simulink model "PW_SMRv10"  (R2022b)
settings: Solver=VariableStepAuto  StartTime=0.0  StopTime=3600 * 5  RelTol=1e-3
libraries: nesl_utility x117, fl_lib x83, SimscapeFluids_lib x11, ee_lib x9, slpidlib x7, simulink x1
(part 1 of 2)
settings Model: Creator=cheap  LastModifiedBy=cheap

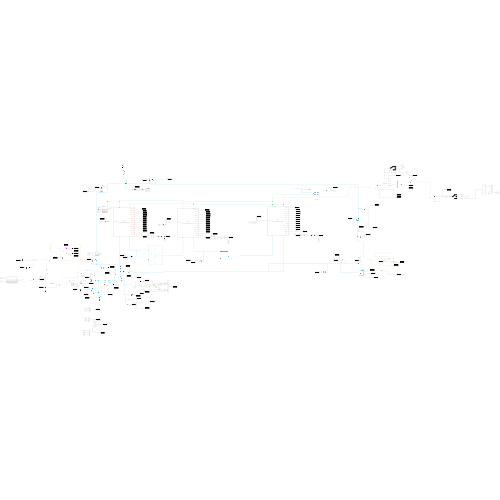
[thumbnail: Simulink's stored preview of the top-level diagram]
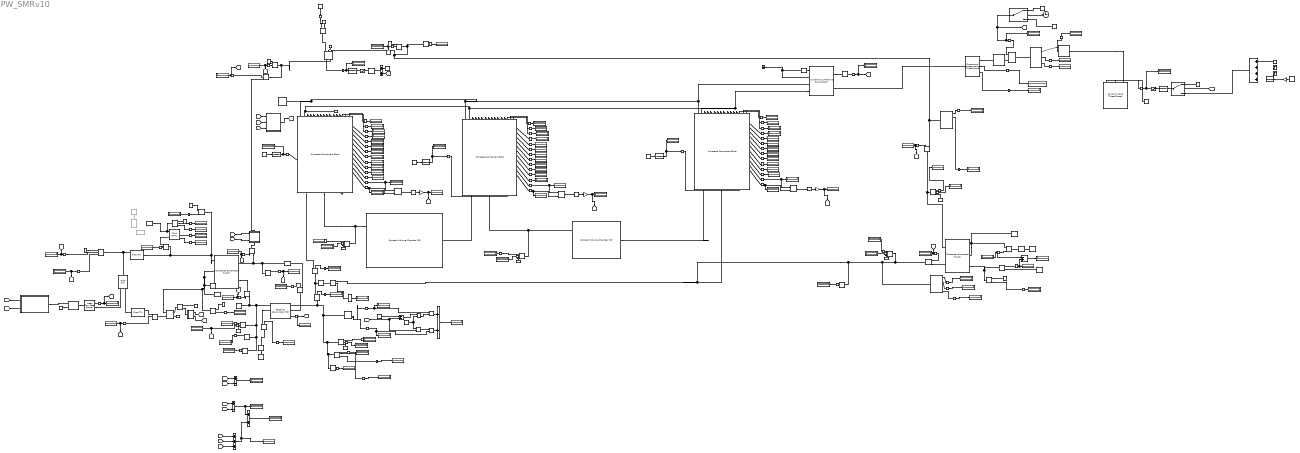
== system PW_SMRv10 ==
  Abs : Abs  SaturateOnIntegerOverflow=off
  Abs1 : Abs  SaturateOnIntegerOverflow=off
  Abs2 : Abs  SaturateOnIntegerOverflow=off
  Absolute Reference (2P){,1..7} (8 alike) : fl_lib/Two-Phase Fluid/Elements/Absolute Reference (2P)
  Absolute Reference (G) : fl_lib/Gas/Elements/Absolute Reference (G)
      settings: InternalSimscapePortConfiguration="{\"Bottom\":[],\"Left\":[{\"id\":\"A\",\"label\":\"\",\"type\":\"foundation.gas.gas\"}],\"Right\":[],\"Top\":[]}"
  Absolute Reference (TL){,1..3} (4 alike) : fl_lib/Thermal Liquid/Elements/Absolute Reference (TL)
  Add : Sum  Inputs=++++
  Add1 : Sum
  Add2 : Sum
  Add3 : Sum  Inputs=+++
  Band-Limited White Noise : simulink/Sources/Band-Limited White Noise  Cov=[0.01]  Ts=0.01  seed=[23341]
  Centrifugal Pump (TL) : SimscapeFluids_lib/Thermal Liquid/Pumps & Motors/Centrifugal Pump (TL)  pump_parameterization=fluids.thermal_liquid.pumps_motors.enum.CentrifugalPumpParameterization.Nominal  capacity_ref_nominal=1670 lpm  head_ref_nominal=40 m  power_ref_nominal=5.6 kW  head_ref_max=60 m  capacity_ref_max=2500 lpm  omega_ref_analytic=376.99 rad/s  flow_rate_1D_TLU=[16.67, 30, 40, 53.33, 66.67, 83.33] lpm  head_1D_TLU=[50, 47.5, 45, 40, 35, 25] m  power_1D_TLU=[.6, .75, .85, .93, .98, .99] kW  omega_ref_1D=3500 rpm  rho_ref_1D=998.21 kg/m^3  flow_rate_2D_TLU=[16.67, 23.33, 30, 40, 53.33, 60] lpm  omega_2D_TLU=[2450, 2800, 3150, 3500] rpm  head_2D_TLU=[25, 32.7, 42.5, 50; 24, 31.7, 41, 49; 22.7, 30.5, 39, 47.5; 20, 28, 36, 45; 15.7, 24, 32, 40; 12.5, 21, 29.5, 37.5] m  power_2D_TLU=[.28, .38, .5, .6; .31, .41, .55, .68; .33, .44, .6, .75; .36, .48, .65, .83; .38, .53, .72, .93; .39, .55, .75, .97] kW  rho_ref_2D=998.21 kg/m^3  diameter_ratio=1  mech_orientation=fluids.thermal_liquid.pumps_motors.enum.CentrifugalPumpMechOrientation.Positive  area=4.56E-3 m^2
      settings: InternalSimscapePortConfiguration="{\"Bottom\":[],\"Left\":[{\"id\":\"A\",\"label\":\"A\",\"type\":\"foundation.thermal_liquid.thermal_liquid\"},{\"id\":\"B\",\"label\":\"B\",\"type\":\"foundation.thermal_liquid.thermal_liquid\"}],\"Right\":[{\"id\":\"R\",\"label\":\"R\",\"type\":\"foundation.mechanical.rotational.rotational\"},{\"id\":\"C\",\"label\":\"C\",\"type\":\"foundation.mechanical.rotational.rotational\"}],\"Top\":[]}"
  Check Valve (2P)2 : SimscapeFluids_lib/Two-Phase Fluid/Valves & Orifices/Directional Control Valves/Check Valve (2P)  opening_pressure_spec=fluids.two_phase_fluid.valves_orifices.enum.PressureControlSpec.Differential  p_crack_differential=0.01 MPa  p_crack_gauge=0.1 MPa  p_max_differential=0.03 MPa  p_max_gauge=0.2 MPa  mdot_nominal_max=0.5 kg/s  delta_p_nominal_max=0.001 MPa  energy_spec=foundation.enum.energy_spec.temperature  p_inlet=5 MPa  T_inlet=225 degC  x_inlet=0.5  alpha_inlet=0.5  h_inlet=1500 kJ/kg  u_inlet=1500 kJ/kg  area=2e-3 m^2  mdot_leak_fraction=2e-3  smoothing_factor=0.01  B_lam=0.999  tau_x=0.1 s
      settings: InternalSimscapePortConfiguration="{\"Bottom\":[],\"Left\":[{\"id\":\"A\",\"label\":\"A\",\"type\":\"foundation.two_phase_fluid.two_phase_fluid\"}],\"Right\":[{\"id\":\"B\",\"label\":\"B\",\"type\":\"foundation.two_phase_fluid.two_phase_fluid\"}],\"Top\":[]}"
  Circuit Breaker (Three-Phase) : ee_lib/Switches & Breakers/Circuit Breaker (Three-Phase)  R_closed=0.001 Ohm  G_open=1e-6 1/Ohm  threshold=0.5 V  breaker_behavior=ee.enum.switches.breakerBehavior.zeroCrossingEnable
      settings: InternalSimscapePortConfiguration="{\"Bottom\":[],\"Left\":[{\"id\":\"vT\",\"label\":\"vT\",\"type\":\"input\"},{\"id\":\"N1\",\"label\":\"~1\",\"type\":\"foundation.electrical.three_phase\"}],\"Right\":[{\"id\":\"N2\",\"label\":\"~2\",\"type\":\"foundation.electrical.three_phase\"}],\"Top\":[]}"
  Clock : Clock
  Condenser : SimscapeFluids_lib/Fluid Network Interfaces/Heat Exchangers/Condenser Evaporator (TL-2P)  flow_arrangement=fluids.interfaces.heat_exchangers.enum.FlowArrangementTL2P.Counter  cross_flow_arrangement=fluids.interfaces.heat_exchangers.enum.CrossFlowArrangementTL2P.MixedUnmixed  R_wall=0 K/kW  area_A1=((1.5*pi)^2)/4 in^2  area_B1=((1.5*pi)^2)/4 in^2  area_A2=6.03e-3 m^2  area_B2=2.03e-3 m^2  flow_geometry_TL=fluids.interfaces.heat_exchangers.enum.FlowGeometryTL.AcrossTubeBank  tube_num_TL=25  tube_length_TL=1 m  tube_cross_section_TL=fluids.interfaces.heat_exchangers.enum.TubeCrossSection.Circular  tube_diameter_TL=0.05 m  tube_width_TL=0.05 m  tube_height_TL=0.05 m  tube_inner_diameter_TL=0.05 m  tube_outer_diameter_TL=0.1 m  tube_flow_area_TL=0.002 m^2  tube_wetted_perimeter_TL=0.15 m  tube_heat_perimeter_TL=0.15 m  tube_pressure_loss_spec_TL=fluids.interfaces.heat_exchangers.enum.TubePressureLossSpec.Haaland  tube_loss_coeff_TL=10  tube_length_add_TL=0.1 m  tube_roughness_pressure_TL=15e-6 m  tube_Re_lam_pressure_TL=2000  tube_Re_tur_pressure_TL=4000  tube_shape_factor_generic_TL=64  tube_heat_coeff_spec_TL=fluids.interfaces.heat_exchangers.enum.TubeHeatCoeffSpec.Gneilinski  tube_colburn_coeff_TL=[.023, .8, .33]  tube_roughness_heat_TL=15e-6 m  tube_Re_lam_heat_TL=2000  tube_Re_tur_heat_TL=4000  tube_Nu_lam_generic_TL=3.66  bank_arrangement_TL=fluids.interfaces.heat_exchangers.enum.BankArrangement.Staggered  bank_num_rows_TL=10  bank_tubes_per_row_TL=10  bank_width_TL=1.5 m  bank_tube_diameter_TL=0.022 m  bank_longitudinal_pitch_TL=0.035 m  bank_transverse_pitch_TL=0.035 m  bank_pressure_loss_spec_TL=fluids.interfaces.heat_exchangers.enum.BankPressureLossSpec.Martin  bank_euler_TL=10  bank_heat_coeff_spec_TL=fluids.interfaces.heat_exchangers.enum.BankHeatCoeffSpec.Martin  bank_colburn_coeff_TL=[.27, .63, .36]  generic_flow_area_TL=0.01 m^2  generic_heat_area_TL=2 m^2  generic_volume_TL=0.05 m^3  generic_loss_coeff_TL=10  generic_colburn_coeff_TL=[.023, .8, .33]  fouling_factor_TL=0 K*m^2/kW  fin_area_TL=0 m^2  fin_efficiency_TL=0.5  p_init_TL=0.2 MPa  T_init_TL=20 degC  tube_num_2P=260  tube_length_2P=1.5 m  tube_cross_section_2P=fluids.interfaces.heat_exchangers.enum.TubeCrossSection.Circular  tube_diameter_2P=0.02 m  tube_width_2P=0.05 m  tube_height_2P=0.05 m  tube_inner_diameter_2P=0.05 m  tube_outer_diameter_2P=0.1 m  tube_flow_area_2P=0.002 m^2  tube_wetted_perimeter_2P=0.15 m  tube_heat_perimeter_2P=0.15 m  tube_pressure_loss_spec_2P=fluids.interfaces.heat_exchangers.enum.TubePressureLossSpec2P.Haaland  tube_loss_coeff_2P=10  tube_length_add_2P=0.1 m  tube_roughness_pressure_2P=15e-6 m  tube_Re_lam_pressure_2P=2000  tube_Re_tur_pressure_2P=4000  tube_shape_factor_generic_2P=64  tube_heat_coeff_spec_2P=fluids.interfaces.heat_exchangers.enum.TubeHeatCoeffSpec2P.GneilinskiCavalliniZecchin  tube_colburn_coeff_liq_2P=[.023, .8, .33]  tube_colburn_coeff_mix_2P=[.05, .8, .33]  tube_colburn_coeff_vap_2P=[.023, .8, .33]  tube_roughness_heat_2P=15e-6 m  tube_Re_lam_heat_2P=2000  tube_Re_tur_heat_2P=4000  tube_Nu_lam_generic_2P=3.66  fouling_factor_2P=0 K*m^2/kW  fin_area_2P=0 m^2  fin_efficiency_2P=0.5  energy_spec_2P=foundation.enum.energy_spec.temperature  p_init_2P=2.5 MPa  T_init_2P=180 degC  x_init_2P=0.5  alpha_init_2P=0.5  h_init_2P=168 kJ/kg  u_init_2P=1500 kJ/kg
      settings: InternalSimscapePortConfiguration="{\"Bottom\":[],\"Left\":[{\"id\":\"A1\",\"label\":\"A1\",\"type\":\"foundation.thermal_liquid.thermal_liquid\"},{\"id\":\"B1\",\"label\":\"B1\",\"type\":\"foundation.thermal_liquid.thermal_liquid\"}],\"Right\":[{\"id\":\"A2\",\"label\":\"A2\",\"type\":\"foundation.two_phase_fluid.two_phase_fluid\"},{\"id\":\"B2\",\"label\":\"B2\",\"type\":\"foundation.two_phase_fluid.two_phase_fluid\"}],\"Top\":[{\"id\":\"Z\",\"label\":\"Z\",\"type\":\"output\"}]}"
  Constant : Constant  Value=1.5
  Constant Volume Chamber (2P) : fl_lib/Two-Phase Fluid/Elements/Constant Volume Chamber (2P)  volume=0.05 m^3  num_ports=foundation.enum.num_ports.two  area_A=5e-2 m^2  area_B=5e-2 m^2  area_C=0.01 m^2  area_D=0.01 m^2  energy_spec=foundation.enum.energy_spec.quality  p_init=3.5 MPa  T_init=293.15 K  x_init=0.85  alpha_init=0.5  h_init=1500 kJ/kg  u_init=1500 kJ/kg  time_constant=0.1 s
      settings: InternalSimscapePortConfiguration="{\"Bottom\":[],\"Left\":[{\"id\":\"A\",\"label\":\"A\",\"type\":\"foundation.two_phase_fluid.two_phase_fluid\"},{\"id\":\"H\",\"label\":\"H\",\"type\":\"foundation.thermal.thermal\"}],\"Right\":[{\"id\":\"B\",\"label\":\"B\",\"type\":\"foundation.two_phase_fluid.two_phase_fluid\"}],\"Top\":[]}"
  Constant Volume Chamber (2P)1 : fl_lib/Two-Phase Fluid/Elements/Constant Volume Chamber (2P)  volume=0.01 m^3  num_ports=foundation.enum.num_ports.two  area_A=5e-2 m^2  area_B=5e-2 m^2  area_C=0.01 m^2  area_D=0.01 m^2  energy_spec=foundation.enum.energy_spec.quality  p_init=1.5 MPa  T_init=293.15 K  x_init=0.85  alpha_init=0.5  h_init=1500 kJ/kg  u_init=1500 kJ/kg  time_constant=0.1 s
      settings: InternalSimscapePortConfiguration="{\"Bottom\":[],\"Left\":[{\"id\":\"A\",\"label\":\"A\",\"type\":\"foundation.two_phase_fluid.two_phase_fluid\"},{\"id\":\"H\",\"label\":\"H\",\"type\":\"foundation.thermal.thermal\"}],\"Right\":[{\"id\":\"B\",\"label\":\"B\",\"type\":\"foundation.two_phase_fluid.two_phase_fluid\"}],\"Top\":[]}"
  Constant Volume Chamber (G) : fl_lib/Gas/Elements/Constant Volume Chamber (G)  Commented=on  volume=0.01 m^3  num_ports=foundation.enum.num_ports.one  area_A=0.01 m^2  area_B=0.01 m^2  area_C=0.01 m^2  area_D=0.01 m^2  p_I_specify=on  p_I_priority=High  p_I=15 MPa  p_I_nominal_specify=off  p_I_nominal_unit=MPa  p_I_nominal_value=1  T_I_specify=on  T_I_priority=High  T_I=315 degC  T_I_nominal_specify=off  T_I_nominal_unit=K  T_I_nominal_value=1  rho_chamber_specify=off  rho_chamber_priority=None  rho_chamber=1.2 kg/m^3  rho_chamber_nominal_specify=off  rho_chamber_nominal_unit=kg/m^3  rho_chamber_nominal_value=1
      settings: InternalSimscapePortConfiguration="{\"Bottom\":[],\"Left\":[{\"id\":\"A\",\"label\":\"A\",\"type\":\"foundation.gas.gas\"},{\"id\":\"H\",\"label\":\"H\",\"type\":\"foundation.thermal.thermal\"}],\"Right\":[],\"Top\":[]}"
  Constant1 : Constant  Value=10
  Constant10 : Constant  Value=550
  Constant2 : Constant  Value=0
  Constant3 : Constant  Value=1.5
  Constant4 : Constant  Value=0
  Constant5 : Constant
  Constant6 : Constant
  Constant7 : Constant  Value=0.55
  Constant8 : Constant  Value=0.6
  Constant9 : Constant  Value=0.345
  Controlled Heat Flow Rate Source : fl_lib/Thermal/Thermal Sources/Controlled Heat Flow Rate Source
  Current and Voltage Sensor (Three-Phase) : ee_lib/Sensors & Transducers/Current and Voltage Sensor (Three-Phase)  vMeasurementType=ee.enum.vmeasurement.ll  outputUnit=ee.enum.unit.si  SRated=100e6 A*V  VRated=24e3 V  I_specify=off  I_priority=None  I=[0, 0, 0] A  I_nominal_specify=off  I_nominal_unit=A  I_nominal_value=1  V_specify=off  V_priority=None  V=[0, 0, 0] V  V_nominal_specify=off  V_nominal_unit=V  V_nominal_value=1
      settings: InternalSimscapePortConfiguration="{\"Bottom\":[],\"Left\":[{\"id\":\"N1\",\"label\":\"~1\",\"type\":\"foundation.electrical.three_phase\"}],\"Right\":[{\"id\":\"V_output\",\"label\":\"V\",\"type\":\"output\"},{\"id\":\"I_output\",\"label\":\"I\",\"type\":\"output\"},{\"id\":\"N2\",\"label\":\"~2\",\"type\":\"foundation.electrical.three_phase\"}],\"Top\":[]}"
  Current and Voltage Sensor (Three-Phase)1 : ee_lib/Sensors & Transducers/Current and Voltage Sensor (Three-Phase)  vMeasurementType=ee.enum.vmeasurement.ll  outputUnit=ee.enum.unit.si  SRated=100e6 A*V  VRated=24e3 V  I_specify=off  I_priority=None  I=[0, 0, 0] A  I_nominal_specify=off  I_nominal_unit=A  I_nominal_value=1  V_specify=off  V_priority=None  V=[0, 0, 0] V  V_nominal_specify=off  V_nominal_unit=V  V_nominal_value=1
      settings: InternalSimscapePortConfiguration="{\"Bottom\":[],\"Left\":[{\"id\":\"N1\",\"label\":\"~1\",\"type\":\"foundation.electrical.three_phase\"}],\"Right\":[{\"id\":\"V_output\",\"label\":\"V\",\"type\":\"output\"},{\"id\":\"I_output\",\"label\":\"I\",\"type\":\"output\"},{\"id\":\"N2\",\"label\":\"~2\",\"type\":\"foundation.electrical.three_phase\"}],\"Top\":[]}"
  DC Voltage Source : fl_lib/Electrical/Electrical Sources/DC Voltage Source  v0=10 V
  Discrete Transfer Fcn{,1..5} (6 alike) : DiscreteTransferFcn  Numerator=[0.18127]  Denominator=[1 -0.81873]
  Discrete PID Controller : slpidlib/PID Controller  Controller=PI  Form=Parallel  TimeDomain=Discrete-time  UseExternalTs=off  SampleTime=-1  IntegratorMethod=Forward Euler  FilterMethod=Forward Euler  ControllerParametersSource=internal  P=1  I=0.05  UseKiTs=off  D=0  N=100  UseFilter=on  TunerSelectOption=Transfer Function Based (PID Tuner App)  InitialConditionSource=internal  InitialConditionForIntegrator=8.33e-6  InitialConditionForFilter=0  DifferentiatorICPrevScaledInput=0  ExternalReset=none  TrackingMode=off  Kt=1  LimitOutput=on  SatLimitsSource=internal  UpperSaturationLimit=8.33e-6 * 4  LowerSaturationLimit=8.33e-6  LinearizeAsGain=off  AntiWindupMode=clamping  Kb=1  LimitIntegrator=off  UpperIntegratorSaturationLimit=inf  LowerIntegratorSaturationLimit=-inf  POutMin=[]  POutMax=[]  IOutMin=[]  IOutMax=[]  DOutMin=[]  DOutMax=[]  NOutMin=[]  NOutMax=[]  SumOutMin=[]  SumOutMax=[]  SaturationOutMin=[]  SaturationOutMax=[]  PParamMin=[]  PParamMax=[]  IParamMin=[]  IParamMax=[]  DParamMin=[]  DParamMax=[]  NParamMin=[]  NParamMax=[]  KbParamMin=[]  KbParamMax=[]  KtParamMin=[]  KtParamMax=[]  KbOutMin=[]  KbOutMax=[]  KtOutMin=[]  KtOutMax=[]  IntegratorOutMin=[]  IntegratorOutMax=[]  FilterOutMin=[]  FilterOutMax=[]  SumI1OutMin=[]  SumI1OutMax=[]  SumI2OutMin=[]  SumI2OutMax=[]  SumI3OutMin=[]  SumI3OutMax=[]  SumI4OutMin=[]  SumI4OutMax=[]  SumDOutMin=[]  SumDOutMax=[]  DifferentiatorOutMin=[]  DifferentiatorOutMax=[]  FilterDiffOutCoefMin=[]  FilterDiffOutCoefMax=[]  ReciprocalOutMin=[]  ReciprocalOutMax=[]  SumDenOutMin=[]  SumDenOutMax=[]  SumNumOutMin=[]  SumNumOutMax=[]  DivideOutMin=[]  DivideOutMax=[]  UdiffTsProdOutMin=[]  UdiffTsProdOutMax=[]  NTsProdOutMin=[]  NTsProdOutMax=[]  UintegralTsProdOutMin=[]  UintegralTsProdOutMax=[]  UngainTsProdOutMin=[]  UngainTsProdOutMax=[]  ClampingZeroOutDataTypeStr=Inherit: Inherit via back propagation  ClampingZeroOutMin=[]  ClampingZeroOutMax=[]  FilterDenConstantOutDataTypeStr=Inherit: Inherit via back propagation  FilterDenConstantOutMin=[]  FilterDenConstantOutMax=[]  PCopyOutDataTypeStr=Inherit: Inherit via back propagation  PCopyOutMin=[]  PCopyOutMax=[]  NCopyOutDataTypeStr=Inherit: Inherit via back propagation  NCopyOutMin=[]  NCopyOutMax=[]  IntegratorContinuousStateAttributes=''  IntegratorStateMustResolveToSignalObject=off  IntegratorRTWStateStorageClass=Auto  FilterContinuousStateAttributes=''  FilterStateMustResolveToSignalObject=off  FilterRTWStateStorageClass=Auto  ParallelPVariant=InternalParameters  IdealPVariant=Disabled  IVariant=InternalParameters  DVariant=Disabled  IntegratorVariant=Discrete  SatVariant=Enabled  AWVariant=DiscClampingParallel  PCopyVariant=Disabled  TRVariant=Disabled  FdbkBlocksVariant=Forward  IdealPFdbkVariant=Disabled  SatFdbkVariant=Disabled  DerivativeFilterVariant=Disabled  NVariant=Disabled  NCopyVariant=Disabled_SignalSpec  FilterICVariant=Disabled  IntegratorICVariant=InternalICs  ExternalResetVariant=Disabled  TRSumVariant=Passthrough  SumFdbkVariant=Disabled  SumVariant=Sum_PI  TsampFilterVariant=InternalTs  TsampNgainVariant=Passthrough  TsampIntegralVariant=Passthrough  ExternalSaturationOutDataTypeStr=Inherit: Same as second input
      settings: LibrarySourceBlock=simulink/Discrete/Discrete PID Controller
  Display{,1..114} (115 alike) : Display
  Dynamic Load (Three-Phase) : ee_lib/Passive/Dynamic Load (Three-Phase)  Vline_rms_min=100 V  Pmin=1e-3 W  enable_fault=simscape.enum.onoff.off  fault_action=simscape.enum.assert.action.none  t_fault=1 s  open_conductance=1e-4 S
      settings: InternalSimscapePortConfiguration="{\"Bottom\":[],\"Left\":[{\"id\":\"N\",\"label\":\"~\",\"type\":\"foundation.electrical.three_phase\"}],\"Right\":[],\"Top\":[{\"id\":\"P\",\"label\":\"P\",\"type\":\"input\"},{\"id\":\"Q\",\"label\":\"Q\",\"type\":\"input\"}]}"
  Electrical Reference : fl_lib/Electrical/Electrical Elements/Electrical Reference
  Gain : Gain  Gain=200
  Gain1 : Gain  Gain=1/1000
  Gain2 : Gain  Gain=1/1000
  Gain3 : Gain  Gain=1/1000
  Gas Properties (G) : fl_lib/Gas/Utilities/Gas Properties (G)  gas_spec=foundation.enum.gas_spec.real_gas  R=0.287 kJ/(K*kg)  Z=1  T_ref=293.15 K  h_ref=420 kJ/kg  cp_ref=1 kJ/(K*kg)  mu_ref=18 s*uPa  k_ref=26 mW/(K*m)  T_TLU1=[150 : 10 : 200, 250 : 50 : 1000, 1500, 2000]' K  h_TLU1=[275.264783730547; 285.377054177734; 295.474578903607; 305.560871069627; 315.638490783961; 325.709373787179; 376.008033649461; 426.297784741196; 476.678788323875; 527.253890684429; 578.12722735187; 629.395040865183; 681.137690131207; 733.415442873049; 786.267894376777; 839.715851152006; 893.764459999509; 948.406676876931; 1003.62653219711; 1059.40193232821; 1115.70691941005; 1172.51341226958; 1762.18512007361; 2377.14064127409] kJ/kg  cp_TLU1=[1.01211492398124; 1.01042105529234; 1.00914159006373; 1.00815898273273; 1.00739688341918; 1.00680484569075; 1.00554191216852; 1.00637389921747; 1.0092105862442; 1.01414404435034; 1.02111299587909; 1.02986878923959; 1.04003820504128; 1.05120320041448; 1.06296312852444; 1.07497111709439; 1.08694865668905; 1.0986858495625; 1.11003396604319; 1.12089493621399; 1.13121051694521; 1.14095251451866; 1.21001953144; 1.24628356718428] kJ/(K*kg)  mu_TLU1=[10.3766056544352; 10.9908682444892; 11.5932000841352; 12.1841060353213; 12.764067709023; 13.3335437107148; 16.038149065057; 18.5373404836509; 20.8671495114253; 23.0554226800681; 25.1239717991959; 27.0901379793485; 28.96790749834; 30.7687111230031; 32.5020036481173; 34.17569027566; 35.7964450415303; 37.3699520751368; 38.9010908824946; 40.3940804368247; 41.8525925389218; 43.279841956487; 56.3254722619962; 68.068290080945] s*uPa  k_TLU1=[14.1517155766309; 15.0474512994325; 15.9300520513026; 16.7998749295306; 17.6573089963228; 18.5027588910197; 22.5644026699512; 26.384465676638; 30.0032801168886; 33.4532006033488; 36.7600619429332; 39.9446251241844; 43.0237448740114; 46.0112537033799; 48.9186234516389; 51.7554617696538; 54.5298878921773; 57.2488200454925; 59.9181976996146; 62.5431553064749; 65.128159527924; 67.6771186900213; 91.7815514375552; 114.486299090693] mW/(K*m)  T_TLU2=T_N2 K  p_TLU2=P_N2 MPa  rho_TLU2=rho_N2 kg/m^3  s_TLU2=s_N2 kJ/(K*kg)  h_TLU2=h_N2 kJ/kg  cp_TLU2=cp_N2 kJ/(K*kg)  mu_TLU2=mu_N2 s*uPa  k_TLU2=k_N2 mW/(K*m)  beta_TLU2=bulk_N2 MPa  alpha_TLU2=beta_N2 1/K  T_min_perfect=1 K  T_max_perfect=inf K  p_min_perfect=1 Pa  p_max_perfect=inf MPa  T_range_flag=foundation.enum.T_range_G.from_props  T_min_semiperfect=150 K  T_max_semiperfect=2000 K  p_min_semiperfect=1 Pa  p_max_semiperfect=inf MPa  pT_region_flag=foundation.enum.pT_region_G.from_props  pT_validity_TLU2=ones(24, 20)  T_min_real=150 K  T_max_real=2000 K  p_min_real=0.001 MPa  p_max_real=10 MPa  p_atm=10 MPa  Mach_rev=0.001
  Heat Flow Rate Sensor : fl_lib/Thermal/Thermal Sensors/Heat Flow Rate Sensor
  Heat Removed : Display
  Ideal Angular Velocity Source : fl_lib/Mechanical/Mechanical Sources/Ideal Angular Velocity Source
  Ideal Angular Velocity Source1 : fl_lib/Mechanical/Mechanical Sources/Ideal Angular Velocity Source
  Local Restriction (TL) : fl_lib/Thermal Liquid/Elements/Local Restriction (TL)  Commented=on  restriction_type=foundation.enum.restriction_type.fixed  restriction_area=5e-5 m^2  min_area=1e-10 m^2  max_area=0.005 m^2  area=1.14e-3 m^2  Cd=0.64  pressure_recovery=simscape.enum.onoff.on  Re_c=12
  Machine Inertia : ee_lib/Electromechanical/Mechanical/Machine Inertia  SRated=15e6 A*V  FRated=60 Hz  nPolePairs=1  inertia_option=2  J=27548 kg*m^2  H=3.525 W*s/(A*V)  damper_option=2  D=39.0509 N*m*s/rad  pu_D=0.12  initialization_option=2  fMechanical0=60 Hz  fElectrical0=60 Hz
      settings: InternalSimscapePortConfiguration="{\"Bottom\":[],\"Left\":[{\"id\":\"R\",\"label\":\"R\",\"type\":\"foundation.mechanical.rotational.rotational\"}],\"Right\":[],\"Top\":[]}"
  Mass & Energy Flow Rate Sensor (2P){,1..9} (10 alike) : fl_lib/Two-Phase Fluid/Sensors/Mass & Energy Flow Rate Sensor (2P)
      settings: InternalSimscapePortConfiguration="{\"Bottom\":[],\"Left\":[{\"id\":\"A\",\"label\":\"A\",\"type\":\"foundation.two_phase_fluid.two_phase_fluid\"}],\"Right\":[{\"id\":\"B\",\"label\":\"B\",\"type\":\"foundation.two_phase_fluid.two_phase_fluid\"},{\"id\":\"M\",\"label\":\"M\",\"type\":\"output\"},{\"id\":\"PHI\",\"label\":\"Phi\",\"type\":\"output\"}],\"Top\":[]}"
  Mass & Energy Flow Rate Sensor (TL){,1..3} (4 alike) : fl_lib/Thermal Liquid/Sensors/Mass & Energy Flow Rate Sensor (TL)
      settings: InternalSimscapePortConfiguration="{\"Bottom\":[],\"Left\":[{\"id\":\"A\",\"label\":\"A\",\"type\":\"foundation.thermal_liquid.thermal_liquid\"}],\"Right\":[{\"id\":\"B\",\"label\":\"B\",\"type\":\"foundation.thermal_liquid.thermal_liquid\"},{\"id\":\"M\",\"label\":\"M\",\"type\":\"output\"},{\"id\":\"PHI\",\"label\":\"Phi\",\"type\":\"output\"}],\"Top\":[]}"
  Mass Flow Rate Source (TL)1 : fl_lib/Thermal Liquid/Sources/Mass Flow Rate Source (TL)  commanded_mass_flow=10 kg/s  area=((1.5*pi)^2)/4 m^2
      settings: InternalSimscapePortConfiguration="{\"Bottom\":[],\"Left\":[{\"id\":\"A\",\"label\":\"A\",\"type\":\"foundation.thermal_liquid.thermal_liquid\"}],\"Right\":[{\"id\":\"B\",\"label\":\"B\",\"type\":\"foundation.thermal_liquid.thermal_liquid\"}],\"Top\":[]}"
  Mechanical Rotational Reference{,1..4} (5 alike) : fl_lib/Mechanical/Rotational Elements/Mechanical Rotational Reference
  PS Constant1 : fl_lib/Physical Signals/Sources/PS Constant  constant=0 kW
  PS-Simulink Converter{,2,14,18,20,22,79,96,101} (9 alike) : nesl_utility/PS-Simulink Converter  PhysicalDomain=network_engine_domain  SubClassName=ps_output  LeftPortType=input  RightPortType=output  PseudoPeriodic=off  Frequencies=[]  VectorFormat=inherit  Unit=MPa  AffineConversion=off
  PS-Simulink Converter{1,3,7,16,24,27,38,45..46,72,81,89,102} (13 alike) : nesl_utility/PS-Simulink Converter  PhysicalDomain=network_engine_domain  SubClassName=ps_output  LeftPortType=input  RightPortType=output  PseudoPeriodic=off  Frequencies=[]  VectorFormat=inherit  Unit=degC  AffineConversion=on
  PS-Simulink Converter10 : nesl_utility/PS-Simulink Converter  PhysicalDomain=network_engine_domain  SubClassName=ps_output  LeftPortType=input  RightPortType=output  PseudoPeriodic=off  Frequencies=[]  VectorFormat=inherit  Unit=MW  AffineConversion=on
  PS-Simulink Converter{4,9,23,54..55,58,64,100} (8 alike) : nesl_utility/PS-Simulink Converter  PhysicalDomain=network_engine_domain  SubClassName=ps_output  LeftPortType=input  RightPortType=output  PseudoPeriodic=off  Frequencies=[]  VectorFormat=inherit  Unit=kg/s  AffineConversion=off
  PS-Simulink Converter{8,11,17,32,99} (5 alike) : nesl_utility/PS-Simulink Converter  PhysicalDomain=network_engine_domain  SubClassName=ps_output  LeftPortType=input  RightPortType=output  PseudoPeriodic=off  Frequencies=[]  VectorFormat=inherit  Unit=1  AffineConversion=off
  PS-Simulink Converter{5,12..13,30..31,33..35,37,40..44,48..53,56..57,65..69,71,73..77,82..86,88,90..94,98} (45 alike) : nesl_utility/PS-Simulink Converter  PhysicalDomain=network_engine_domain  SubClassName=ps_output  LeftPortType=input  RightPortType=output  PseudoPeriodic=off  Frequencies=[]  VectorFormat=inherit  Unit=inherit  AffineConversion=off
  PS-Simulink Converter{6,15,19,21,80,97} (6 alike) : nesl_utility/PS-Simulink Converter  PhysicalDomain=network_engine_domain  SubClassName=ps_output  LeftPortType=input  RightPortType=output  PseudoPeriodic=off  Frequencies=[]  VectorFormat=inherit  Unit=kJ/kg  AffineConversion=off
  PS-Simulink Converter25 : nesl_utility/PS-Simulink Converter  PhysicalDomain=network_engine_domain  SubClassName=ps_output  LeftPortType=input  RightPortType=output  PseudoPeriodic=off  Frequencies=[]  VectorFormat=inherit  Unit=kJ/kg  AffineConversion=on
  PS-Simulink Converter26 : nesl_utility/PS-Simulink Converter  PhysicalDomain=network_engine_domain  SubClassName=ps_output  LeftPortType=input  RightPortType=output  PseudoPeriodic=off  Frequencies=[]  VectorFormat=inherit  Unit=kJ/kg  AffineConversion=on
  PS-Simulink Converter28 : nesl_utility/PS-Simulink Converter  PhysicalDomain=network_engine_domain  SubClassName=ps_output  LeftPortType=input  RightPortType=output  PseudoPeriodic=off  Frequencies=[]  VectorFormat=inherit  Unit=kJ/kg  AffineConversion=on
  PS-Simulink Converter{29,59..63} (6 alike) : nesl_utility/PS-Simulink Converter  PhysicalDomain=network_engine_domain  SubClassName=ps_output  LeftPortType=input  RightPortType=output  PseudoPeriodic=off  Frequencies=[]  VectorFormat=inherit  Unit=kW  AffineConversion=on
  PS-Simulink Converter36 : nesl_utility/PS-Simulink Converter  PhysicalDomain=network_engine_domain  SubClassName=ps_output  LeftPortType=input  RightPortType=output  PseudoPeriodic=off  Frequencies=[]  VectorFormat=inherit  Unit=m^2  AffineConversion=on
  PS-Simulink Converter39 : nesl_utility/PS-Simulink Converter  PhysicalDomain=network_engine_domain  SubClassName=ps_output  LeftPortType=input  RightPortType=output  PseudoPeriodic=off  Frequencies=[]  VectorFormat=inherit  Unit=MPa  AffineConversion=on
  PS-Simulink Converter47 : nesl_utility/PS-Simulink Converter  PhysicalDomain=network_engine_domain  SubClassName=ps_output  LeftPortType=input  RightPortType=output  PseudoPeriodic=off  Frequencies=[]  VectorFormat=inherit  Unit=rad/s  AffineConversion=on
  PS-Simulink Converter70 : nesl_utility/PS-Simulink Converter  PhysicalDomain=network_engine_domain  SubClassName=ps_output  LeftPortType=input  RightPortType=output  PseudoPeriodic=off  Frequencies=[]  VectorFormat=inherit  Unit=m^2  AffineConversion=on
  PS-Simulink Converter78 : nesl_utility/PS-Simulink Converter  PhysicalDomain=network_engine_domain  SubClassName=ps_output  LeftPortType=input  RightPortType=output  PseudoPeriodic=off  Frequencies=[]  VectorFormat=inherit  Unit=rad/s  AffineConversion=on
  PS-Simulink Converter87 : nesl_utility/PS-Simulink Converter  PhysicalDomain=network_engine_domain  SubClassName=ps_output  LeftPortType=input  RightPortType=output  PseudoPeriodic=off  Frequencies=[]  VectorFormat=inherit  Unit=m^2  AffineConversion=on
  PS-Simulink Converter95 : nesl_utility/PS-Simulink Converter  PhysicalDomain=network_engine_domain  SubClassName=ps_output  LeftPortType=input  RightPortType=output  PseudoPeriodic=off  Frequencies=[]  VectorFormat=inherit  Unit=rad/s  AffineConversion=on
  Pipe (TL) : fl_lib/Thermal Liquid/Elements/Pipe (TL)  length=3 m  area=4.56E-3 m^2  Dh=1.5 in  length_add=1 m  roughness=15e-6 m  Re_lam=2000  Re_tur=4000  shape_factor=64  Nu_lam=3.66  dynamic_compressibility=simscape.enum.onoff.on  inertia=simscape.enum.onoff.off  p0=15 MPa  T0=300 degC  mdot0=0 kg/s
  Pipe (TL)1 : fl_lib/Thermal Liquid/Elements/Pipe (TL)  length=6 m  area=4.56E-3 m^2  Dh=1.5 in  length_add=1 m  roughness=15e-6 m  Re_lam=2000  Re_tur=4000  shape_factor=64  Nu_lam=3.66  dynamic_compressibility=simscape.enum.onoff.on  inertia=simscape.enum.onoff.off  p0=15 MPa  T0=300 degC  mdot0=0 kg/s
  Pipe (TL)2 : fl_lib/Thermal Liquid/Elements/Pipe (TL)  length=6 m  area=4.56E-3 m^2  Dh=1.5 in  length_add=1 m  roughness=15e-6 m  Re_lam=2000  Re_tur=4000  shape_factor=64  Nu_lam=3.66  dynamic_compressibility=simscape.enum.onoff.on  inertia=simscape.enum.onoff.off  p0=15 MPa  T0=300 degC  mdot0=0 kg/s
  Power Sensor (Three-Phase) : ee_lib/Sensors & Transducers/Power Sensor (Three-Phase)  load_type=ee.enum.passive.type_balanced.balanced  f0=60 Hz  config=ee.enum.with_neutral.no  rho=1
      settings: InternalSimscapePortConfiguration="{\"Bottom\":[],\"Left\":[{\"id\":\"N1\",\"label\":\"~1\",\"type\":\"foundation.electrical.three_phase\"}],\"Right\":[{\"id\":\"N2\",\"label\":\"~2\",\"type\":\"foundation.electrical.three_phase\"}],\"Top\":[{\"id\":\"Pm\",\"label\":\"P\",\"type\":\"output\"},{\"id\":\"Qm\",\"label\":\"Q\",\"type\":\"output\"}]}"
  Preheating : Subsystem
      settings: PortSchema="{\"entries\":[{\"content\":{\"sides\":[{\"content\":{\"connectorIds\":[\"In1\",\"In2\",\"In3\"]},\"type\":\"ConnectorPlacement.EquallySpacedRectSide\",\"uuid\":\"32777bd1-5361-468e-8441-a7542eaf585a\"},{\"content\":{\"connectorIds\":[],\"side\":\"RIGHT\"},\"type\":\"ConnectorPlacement.EquallySpacedRectSide\",\"uuid\":\"4d6640a9-62f4-4987-a198-57008f8c132c\"},{\"content\":{\"connectorIds\":[\"LConn1\"],\"side\":\"TOP\"},\"type\":\"ConnectorPlacement.EquallySpacedRectSide\",\"uuid\":\"666f6154-3a6e-49f7-b11f-a7175ac46304\"},{\"content\":{\"connectorIds\":[\"RConn1\"],\"side\":\"BOTTOM\"},\"type\":\"ConnectorPlacement.EquallySpacedRectSide\",\"uuid\":\"f7a22bed-9308-40d7-99fb-c8a013123d35\"}]},\"type\":\"ConnectorPlacement.EquallySpacedConnector\",\"uuid\":\"3a4891e5-e5f0-4b84-878d-e1460854c778\"}],\"packageUris\":[\"http://schema.mathworks.com/mf0/Connector/R2020b\"],\"version\":\"1.0\"}"
  Pressure & Temperature Sensor (G) : fl_lib/Gas/Sensors/Pressure & Temperature Sensor (G)
      settings: InternalSimscapePortConfiguration="{\"Bottom\":[],\"Left\":[{\"id\":\"A\",\"label\":\"A\",\"type\":\"foundation.gas.gas\"}],\"Right\":[{\"id\":\"B\",\"label\":\"B\",\"type\":\"foundation.gas.gas\"},{\"id\":\"P\",\"label\":\"P\",\"type\":\"output\"},{\"id\":\"T\",\"label\":\"T\",\"type\":\"output\"}],\"Top\":[]}"
  Pressure & Temperature Sensor (TL){,1..3} (4 alike) : fl_lib/Thermal Liquid/Sensors/Pressure & Temperature Sensor (TL)
      settings: InternalSimscapePortConfiguration="{\"Bottom\":[],\"Left\":[{\"id\":\"A\",\"label\":\"A\",\"type\":\"foundation.thermal_liquid.thermal_liquid\"}],\"Right\":[{\"id\":\"B\",\"label\":\"B\",\"type\":\"foundation.thermal_liquid.thermal_liquid\"},{\"id\":\"P\",\"label\":\"P\",\"type\":\"output\"},{\"id\":\"T\",\"label\":\"T\",\"type\":\"output\"}],\"Top\":[]}"
  Pressure & Internal Energy Sensor (2P){,1..7} (8 alike) : fl_lib/Two-Phase Fluid/Sensors/Pressure & Internal Energy Sensor (2P)
      settings: InternalSimscapePortConfiguration="{\"Bottom\":[],\"Left\":[{\"id\":\"A\",\"label\":\"A\",\"type\":\"foundation.two_phase_fluid.two_phase_fluid\"}],\"Right\":[{\"id\":\"B\",\"label\":\"B\",\"type\":\"foundation.two_phase_fluid.two_phase_fluid\"},{\"id\":\"P\",\"label\":\"P\",\"type\":\"output\"},{\"id\":\"U\",\"label\":\"U\",\"type\":\"output\"}],\"Top\":[]}"
  Pressure Relief Valve (2P) : SimscapeFluids_lib/Two-Phase Fluid/Valves & Orifices/Pressure Control Valves/Pressure Relief Valve (2P)  set_pressure_control=foundation.enum.constant_controlled.constant  set_pressure_spec=fluids.two_phase_fluid.valves_orifices.enum.PressureControlSpec.Gauge  p_set_differential=0.01 MPa  p_set_gauge=7.5 MPa  p_range=0.1 MPa  mdot_nominal_max=0.5 kg/s  delta_p_nominal_max=3 MPa  energy_spec=foundation.enum.energy_spec.temperature  p_inlet=7 MPa  T_inlet=293.15 degC  x_inlet=0.5  alpha_inlet=0.5  h_inlet=1500 kJ/kg  u_inlet=1500 kJ/kg  area=2e-3 m^2  mdot_leak_fraction=1e-6  smoothing_factor=0.01  B_lam=0.999  tau_x=0.1 s
      settings: InternalSimscapePortConfiguration="{\"Bottom\":[],\"Left\":[{\"id\":\"A\",\"label\":\"A\",\"type\":\"foundation.two_phase_fluid.two_phase_fluid\"}],\"Right\":[{\"id\":\"B\",\"label\":\"B\",\"type\":\"foundation.two_phase_fluid.two_phase_fluid\"}],\"Top\":[]}"
  Pressure Relief Valve (2P)1 : SimscapeFluids_lib/Two-Phase Fluid/Valves & Orifices/Pressure Control Valves/Pressure Relief Valve (2P)  set_pressure_control=foundation.enum.constant_controlled.constant  set_pressure_spec=fluids.two_phase_fluid.valves_orifices.enum.PressureControlSpec.Gauge  p_set_differential=0.01 MPa  p_set_gauge=10 MPa  p_range=0.1 MPa  mdot_nominal_max=0.1 kg/s  delta_p_nominal_max=0.001 MPa  energy_spec=foundation.enum.energy_spec.temperature  p_inlet=7 MPa  T_inlet=280 degC  x_inlet=0.5  alpha_inlet=0.5  h_inlet=1500 kJ/kg  u_inlet=1500 kJ/kg  area=((1.5*pi)^2)/4 in^2  mdot_leak_fraction=1e-6  smoothing_factor=0.01  B_lam=0.999  tau_x=0.1 s
      settings: InternalSimscapePortConfiguration="{\"Bottom\":[],\"Left\":[{\"id\":\"A\",\"label\":\"A\",\"type\":\"foundation.two_phase_fluid.two_phase_fluid\"}],\"Right\":[{\"id\":\"B\",\"label\":\"B\",\"type\":\"foundation.two_phase_fluid.two_phase_fluid\"}],\"Top\":[]}"
  Product{,1..6} (7 alike) : Product
  Qcond : Display
  Qsg : Display
  Reservoir (2P) : fl_lib/Two-Phase Fluid/Elements/Reservoir (2P)  pressure_spec=foundation.enum.ReservoirPressureSpec2P.Specified  reservoir_pressure=4 MPa  reservoir_condensing_temperature=373.15 K  reservoir_evaporating_temperature=373.15 K  energy_spec=foundation.enum.ReservoirEnergySpec2P.Temperature  reservoir_temperature=120 degC  reservoir_quality=0.5  reservoir_void_fraction=0.5  reservoir_enthalpy=483 kJ/kg  reservoir_internal_energy=1500 kJ/kg  reservoir_subcooling=5 deltaK  reservoir_superheating=5 deltaK  area_A=0.01 m^2
  Reservoir (TL) : fl_lib/Thermal Liquid/Elements/Reservoir (TL)  Commented=on  pressure_spec=foundation.enum.pressure_spec.specified  reservoir_pressure=15 MPa  reservoir_temperature=315 degC  area=0.01 m^2
  Reservoir (TL)1 : fl_lib/Thermal Liquid/Elements/Reservoir (TL)  pressure_spec=foundation.enum.pressure_spec.specified  reservoir_pressure=0.2 MPa  reservoir_temperature=20 degC  area=((1.5*pi)^2)/4 in^2
  Reservoir (TL)2 : fl_lib/Thermal Liquid/Elements/Reservoir (TL)  pressure_spec=foundation.enum.pressure_spec.atmospheric  reservoir_pressure=0.2 MPa  reservoir_temperature=20 degC  area=((1.5*pi)^2)/4 in^2
  Saturation : Saturate  UpperLimit=8.33e-6*4  LowerLimit=8.33e-6
  Saturation Properties Sensor (2P) : fl_lib/Two-Phase Fluid/Sensors/Saturation Properties Sensor (2P)  pressure_measure=simscape.enum.onoff.off  pressure_check=simscape.enum.assert.action.error  energy_measure=foundation.enum.EnergyMeasurement.Off  density_measure=foundation.enum.DensityMeasurement.SaturatedDensity
      settings: InternalSimscapePortConfiguration="{\"Bottom\":[{\"id\":\"rho_sat_liq\",\"label\":\"rhoL\",\"type\":\"output\"},{\"id\":\"rho_sat_vap\",\"label\":\"rhoV\",\"type\":\"output\"}],\"Left\":[{\"id\":\"A\",\"label\":\"A\",\"type\":\"foundation.two_phase_fluid.two_phase_fluid\"}],\"Right\":[{\"id\":\"T_sat_liq\",\"label\":\"TL\",\"type\":\"output\"},{\"id\":\"T_sat_vap\",\"label\":\"TV\",\"type\":\"output\"}],\"Top\":[]}"
  Saturation1 : Saturate  UpperLimit=1000  LowerLimit=0
  Simscape Component : SimscapeComponentBlock  SourceFile=custom_turbine_2p_layer4_mechanical_floweff_safe  ComponentPath=custom_turbine_2p_layer4_mechanical_floweff_safe  ComponentVariants="[\"custom_turbine_2p_layer4_mechanical_floweff_safe\"]"  ComponentVariantNames="[\"custom_turbine_2p_layer4_mechanical_floweff_safe\"]"  ClassName=custom_turbine_2p_layer4_mechanical_floweff_safe  SchemaVersion=1  pA_nom=6.5 MPa  pB_nom=1.5 MPa  mdot_nom=1 kg/s  dp_min=1 kPa  omega_min=1 rad/s  nozzle_area_max=4e-4 m^2  nozzle_Cd=0.85  vapor_R=461.5 J/(K*kg)  vapor_gamma=1.30  eta_peak=0.80  mdot_ratio_peak=0.80  efficiency_flow_curve=0.20  p_expansion_min=100 kPa  p_expansion_max=100 MPa  max_enthalpy_drop=500 kJ/kg
      settings: CopyFcn=simscape.engine.sli.internal.componentblockcallback(gcbh,'COPY')  PreCopyFcn=simscape.engine.sli.internal.componentblockcallback(gcbh,'PRECOPY')  PreDeleteFcn=simscape.engine.sli.internal.componentblockcallback(gcbh,'PREDELETE')  InternalSimscapePortConfiguration="{\"Bottom\":[{\"id\":\"shaft_torque_out\",\"label\":\"shaft_torque_out\",\"type\":\"output\"},{\"id\":\"shaft_speed_out\",\"label\":\"shaft_speed_out\",\"type\":\"output\"},{\"id\":\"enthalpy_drop_out\",\"label\":\"enthalpy_drop_out\",\"type\":\"output\"},{\"id\":\"ideal_outlet_quality\",\"label\":\"ideal_outlet_quality\",\"type\":\"output\"},{\"id\":\"ideal_outlet_enthalpy\",\"label\":\"ideal_outlet_enthalpy\",\"type\":\"output\"},{\"id\":\"inlet_entropy\",\"label\":\"inlet_entropy\",\"type\":\"output\"},{\"id\":\"efficiency_out\",\"label\":\"efficiency_out\",\"type\":\"output\"},{\"id\":\"nozzle_opening_out\",\"label\":\"nozzle_opening_out\",\"type\":\"output\"},{\"id\":\"nozzle_area_out\",\"label\":\"nozzle_area_out\",\"type\":\"output\"},{\"id\":\"mass_flow_out\",\"label\":\"mass_flow_out\",\"type\":\"output\"},{\"id\":\"inlet_temperature_out\",\"label\":\"inlet_temperature_out\",\"type\":\"output\"},{\"id\":\"pressure_ratio_out\",\"label\":\"pressure_ratio_out\",\"type\":\"output\"},{\"id\":\"mass_flow_ratio_out\",\"label\":\"mass_flow_ratio_out\",\"type\":\"output\"},{\"id\":\"nozzle_choked_out\",\"label\":\"nozzle_choked_out\",\"type\":\"output\"}],\"Left\":[{\"id\":\"A\",\"label\":\"A\",\"type\":\"foundation.two_phase_fluid.two_phase_fluid\"},{\"id\":\"B\",\"label\":\"B\",\"type\":\"foundation.two_phase_fluid.two_phase_fluid\"}],\"Right\":[{\"id\":\"R\",\"label\":\"R\",\"type\":\"foundation.mechanical.rotational.rotational\"},{\"id\":\"C\",\"label\":\"C\",\"type\":\"foundation.mechanical.rotational.rotational\"}],\"Top\":[{\"id\":\"nozzle_command\",\"label\":\"nozzle_command\",\"type\":\"input\"}]}"
      mask Type: custom_turbine_2p_layer4_mechanical_floweff_safe
  Simscape Component1 : SimscapeComponentBlock  SourceFile=custom_turbine_2p_layer4_mechanical_floweff_safe  ComponentPath=custom_turbine_2p_layer4_mechanical_floweff_safe  ComponentVariants="[\"custom_turbine_2p_layer4_mechanical_floweff_safe\"]"  ComponentVariantNames="[\"custom_turbine_2p_layer4_mechanical_floweff_safe\"]"  ClassName=custom_turbine_2p_layer4_mechanical_floweff_safe  SchemaVersion=1  pA_nom=3.5 MPa  pB_nom=1.5 MPa  mdot_nom=1 kg/s  dp_min=1 kPa  omega_min=1 rad/s  nozzle_area_max=4e-4 m^2  nozzle_Cd=0.85  vapor_R=461.5 J/(K*kg)  vapor_gamma=1.30  eta_peak=0.80  mdot_ratio_peak=0.80  efficiency_flow_curve=0.20  p_expansion_min=100 kPa  p_expansion_max=100 MPa  max_enthalpy_drop=500 kJ/kg
      settings: CopyFcn=simscape.engine.sli.internal.componentblockcallback(gcbh,'COPY')  PreCopyFcn=simscape.engine.sli.internal.componentblockcallback(gcbh,'PRECOPY')  PreDeleteFcn=simscape.engine.sli.internal.componentblockcallback(gcbh,'PREDELETE')  InternalSimscapePortConfiguration="{\"Bottom\":[{\"id\":\"shaft_torque_out\",\"label\":\"shaft_torque_out\",\"type\":\"output\"},{\"id\":\"shaft_speed_out\",\"label\":\"shaft_speed_out\",\"type\":\"output\"},{\"id\":\"enthalpy_drop_out\",\"label\":\"enthalpy_drop_out\",\"type\":\"output\"},{\"id\":\"ideal_outlet_quality\",\"label\":\"ideal_outlet_quality\",\"type\":\"output\"},{\"id\":\"ideal_outlet_enthalpy\",\"label\":\"ideal_outlet_enthalpy\",\"type\":\"output\"},{\"id\":\"inlet_entropy\",\"label\":\"inlet_entropy\",\"type\":\"output\"},{\"id\":\"efficiency_out\",\"label\":\"efficiency_out\",\"type\":\"output\"},{\"id\":\"nozzle_opening_out\",\"label\":\"nozzle_opening_out\",\"type\":\"output\"},{\"id\":\"nozzle_area_out\",\"label\":\"nozzle_area_out\",\"type\":\"output\"},{\"id\":\"mass_flow_out\",\"label\":\"mass_flow_out\",\"type\":\"output\"},{\"id\":\"inlet_temperature_out\",\"label\":\"inlet_temperature_out\",\"type\":\"output\"},{\"id\":\"pressure_ratio_out\",\"label\":\"pressure_ratio_out\",\"type\":\"output\"},{\"id\":\"mass_flow_ratio_out\",\"label\":\"mass_flow_ratio_out\",\"type\":\"output\"},{\"id\":\"nozzle_choked_out\",\"label\":\"nozzle_choked_out\",\"type\":\"output\"}],\"Left\":[{\"id\":\"A\",\"label\":\"A\",\"type\":\"foundation.two_phase_fluid.two_phase_fluid\"},{\"id\":\"B\",\"label\":\"B\",\"type\":\"foundation.two_phase_fluid.two_phase_fluid\"}],\"Right\":[{\"id\":\"R\",\"label\":\"R\",\"type\":\"foundation.mechanical.rotational.rotational\"},{\"id\":\"C\",\"label\":\"C\",\"type\":\"foundation.mechanical.rotational.rotational\"}],\"Top\":[{\"id\":\"nozzle_command\",\"label\":\"nozzle_command\",\"type\":\"input\"}]}"
      mask Type: custom_turbine_2p_layer4_mechanical_floweff_safe
  Simscape Component2 : SimscapeComponentBlock  SourceFile=custom_turbine_2p_layer4_mechanical_floweff_safe  ComponentPath=custom_turbine_2p_layer4_mechanical_floweff_safe  ComponentVariants="[\"custom_turbine_2p_layer4_mechanical_floweff_safe\"]"  ComponentVariantNames="[\"custom_turbine_2p_layer4_mechanical_floweff_safe\"]"  ClassName=custom_turbine_2p_layer4_mechanical_floweff_safe  SchemaVersion=1  pA_nom=1.5 MPa  pB_nom=0.3 MPa  mdot_nom=1 kg/s  dp_min=1 kPa  omega_min=1 rad/s  nozzle_area_max=4e-4 m^2  nozzle_Cd=0.85  vapor_R=461.5 J/(K*kg)  vapor_gamma=1.30  eta_peak=0.80  mdot_ratio_peak=0.80  efficiency_flow_curve=0.20  p_expansion_min=100 kPa  p_expansion_max=100 MPa  max_enthalpy_drop=500 kJ/kg
      settings: CopyFcn=simscape.engine.sli.internal.componentblockcallback(gcbh,'COPY')  PreCopyFcn=simscape.engine.sli.internal.componentblockcallback(gcbh,'PRECOPY')  PreDeleteFcn=simscape.engine.sli.internal.componentblockcallback(gcbh,'PREDELETE')  InternalSimscapePortConfiguration="{\"Bottom\":[{\"id\":\"shaft_torque_out\",\"label\":\"shaft_torque_out\",\"type\":\"output\"},{\"id\":\"shaft_speed_out\",\"label\":\"shaft_speed_out\",\"type\":\"output\"},{\"id\":\"enthalpy_drop_out\",\"label\":\"enthalpy_drop_out\",\"type\":\"output\"},{\"id\":\"ideal_outlet_quality\",\"label\":\"ideal_outlet_quality\",\"type\":\"output\"},{\"id\":\"ideal_outlet_enthalpy\",\"label\":\"ideal_outlet_enthalpy\",\"type\":\"output\"},{\"id\":\"inlet_entropy\",\"label\":\"inlet_entropy\",\"type\":\"output\"},{\"id\":\"efficiency_out\",\"label\":\"efficiency_out\",\"type\":\"output\"},{\"id\":\"nozzle_opening_out\",\"label\":\"nozzle_opening_out\",\"type\":\"output\"},{\"id\":\"nozzle_area_out\",\"label\":\"nozzle_area_out\",\"type\":\"output\"},{\"id\":\"mass_flow_out\",\"label\":\"mass_flow_out\",\"type\":\"output\"},{\"id\":\"inlet_temperature_out\",\"label\":\"inlet_temperature_out\",\"type\":\"output\"},{\"id\":\"pressure_ratio_out\",\"label\":\"pressure_ratio_out\",\"type\":\"output\"},{\"id\":\"mass_flow_ratio_out\",\"label\":\"mass_flow_ratio_out\",\"type\":\"output\"},{\"id\":\"nozzle_choked_out\",\"label\":\"nozzle_choked_out\",\"type\":\"output\"}],\"Left\":[{\"id\":\"A\",\"label\":\"A\",\"type\":\"foundation.two_phase_fluid.two_phase_fluid\"},{\"id\":\"B\",\"label\":\"B\",\"type\":\"foundation.two_phase_fluid.two_phase_fluid\"}],\"Right\":[{\"id\":\"R\",\"label\":\"R\",\"type\":\"foundation.mechanical.rotational.rotational\"},{\"id\":\"C\",\"label\":\"C\",\"type\":\"foundation.mechanical.rotational.rotational\"}],\"Top\":[{\"id\":\"nozzle_command\",\"label\":\"nozzle_command\",\"type\":\"input\"}]}"
      mask Type: custom_turbine_2p_layer4_mechanical_floweff_safe
  Simulink-PS Converter : nesl_utility/Simulink-PS Converter  PhysicalDomain=network_engine_domain  SubClassName=ps_input  LeftPortType=input  RightPortType=output  PseudoPeriodic=off  Frequencies=[]  NoiseDistribution=none  NoiseParameters=[]  Unit=m^3/rev  AffineConversion=off  FilteringAndDerivatives=provide  SimscapeFilterOrder=1  InputFilterTimeConstant=0.001  UdotUserProvided=0
  Simulink-PS Converter1 : nesl_utility/Simulink-PS Converter  PhysicalDomain=network_engine_domain  SubClassName=ps_input  LeftPortType=input  RightPortType=output  PseudoPeriodic=off  Frequencies=[]  NoiseDistribution=none  NoiseParameters=[]  Unit=kW  AffineConversion=off  FilteringAndDerivatives=provide  SimscapeFilterOrder=1  InputFilterTimeConstant=0.001  UdotUserProvided=0
  Simulink-PS Converter2 : nesl_utility/Simulink-PS Converter  PhysicalDomain=network_engine_domain  SubClassName=ps_input  LeftPortType=input  RightPortType=output  PseudoPeriodic=off  Frequencies=[]  NoiseDistribution=none  NoiseParameters=[]  Unit=V  AffineConversion=off  FilteringAndDerivatives=provide  SimscapeFilterOrder=1  InputFilterTimeConstant=0.001  UdotUserProvided=0
  Simulink-PS Converter3 : nesl_utility/Simulink-PS Converter  PhysicalDomain=network_engine_domain  SubClassName=ps_input  LeftPortType=input  RightPortType=output  PseudoPeriodic=off  Frequencies=[]  NoiseDistribution=none  NoiseParameters=[]  Unit=1  AffineConversion=off  FilteringAndDerivatives=provide  SimscapeFilterOrder=1  InputFilterTimeConstant=0.001  UdotUserProvided=0
  Simulink-PS Converter4 : nesl_utility/Simulink-PS Converter  PhysicalDomain=network_engine_domain  SubClassName=ps_input  LeftPortType=input  RightPortType=output  PseudoPeriodic=off  Frequencies=[]  NoiseDistribution=none  NoiseParameters=[]  Unit=1  AffineConversion=off  FilteringAndDerivatives=provide  SimscapeFilterOrder=1  InputFilterTimeConstant=0.001  UdotUserProvided=0
  Simulink-PS Converter5 : nesl_utility/Simulink-PS Converter  PhysicalDomain=network_engine_domain  SubClassName=ps_input  LeftPortType=input  RightPortType=output  PseudoPeriodic=off  Frequencies=[]  NoiseDistribution=none  NoiseParameters=[]  Unit=1  AffineConversion=off  FilteringAndDerivatives=provide  SimscapeFilterOrder=1  InputFilterTimeConstant=0.001  UdotUserProvided=0
  Simulink-PS Converter6 : nesl_utility/Simulink-PS Converter  PhysicalDomain=network_engine_domain  SubClassName=ps_input  LeftPortType=input  RightPortType=output  PseudoPeriodic=off  Frequencies=[]  NoiseDistribution=none  NoiseParameters=[]  Unit=rad/s  AffineConversion=off  FilteringAndDerivatives=provide  SimscapeFilterOrder=1  InputFilterTimeConstant=0.001  UdotUserProvided=0
  Solver Configuration : nesl_utility/Solver Configuration  PhysicalDomain=network_engine_domain  SubClassName=solver  LeftPortType=input  RightPortType=generic  Tones=[]  Harmonics=[]  SimulateNoise=off  Profile=off  UseLocalSampling=off  EnableSwitchedLinearOptims=on  FrequencyDomain=off  UseCCode=off  RelTol=0.001  AbsTol=0.001  MinStep=1e-09  ToWorkspace=off  RevertToSquareIcSolve=off  NumHomotopyIterations=100  PhasorMode=off  PhasorModeNumHarmonics=1  ConsistencySolver=NEWTON_XTOL_AFTER_FTOL  IndexReductionMethod=DerivativeReplacement  DoDC=off  ResidualTolerance=1e-09  ConsistencyTolSource=GLOBAL  ConsistencyAbsTol=0.001  ConsistencyRelTol=0.001  ConsistencyTolFactor=0.01  UseLocalSolver=on  LocalSolverChoice=NE_BACKWARD_EULER_ADVANCER  ResolveIndetEquations=on  FunctionEvalNumThread=1  LocalSolverSampleTime=0.01  DoFixedCost=on  MaxNonlinIter=3  MaxModeIter=2  ComputeImpulses=off  ImpulseIterations=2  LinearAlgebra=auto  LinearAlgebraNumThread=0  EquationFormulation=NE_TIME_EF  DelaysMemoryBudget=1024  AutomaticFiltering=on  FilteringTimeConstant=0.001  PartitionStorageMethod=AS_NEEDED  PartitionMemoryBudget=1024  PartitionMethod=ROBUST
  Startup Controller : Subsystem
  Steam Drum : SimscapeFluids_lib/Two-Phase Fluid/Tanks & Accumulators/Receiver Accumulator (2P)  volume=3 m^3  tank_area=0.5 m^2  area_AV=2e-3 m^2  area_BV=2e-3 m^2  area_AL=((1.5*pi)^2)/4 in^2  area_BL=((1.5*pi)^2)/4 in^2  V_frac_error=simscape.enum.assert.action.none  V_frac_min=0.05  V_frac_max=0.95  V_frac_smooth=0.05  p_crit_error=simscape.enum.assert.action.error  hc_vap=75 W/(K*m^2)  hc_liq=2500 W/(K*m^2)  receiver_accumulator_energy_spec=fluids.two_phase_fluid.enum.receiver_accumulator_energy_spec.volume_fraction  p_init=4 MPa  T_init=280 degC  M_frac_init=0.7  V_frac_init=0.2  h_init=1500 kJ/kg  u_init=1500 kJ/kg  tau_vap_cond=0.1 s
      settings: InternalSimscapePortConfiguration="{\"Bottom\":[],\"Left\":[{\"id\":\"AV\",\"label\":\"AV\",\"type\":\"foundation.two_phase_fluid.two_phase_fluid\"},{\"id\":\"AL\",\"label\":\"AL\",\"type\":\"foundation.two_phase_fluid.two_phase_fluid\"},{\"id\":\"H\",\"label\":\"H\",\"type\":\"foundation.thermal.thermal\"}],\"Right\":[{\"id\":\"BV\",\"label\":\"BV\",\"type\":\"foundation.two_phase_fluid.two_phase_fluid\"},{\"id\":\"BL\",\"label\":\"BL\",\"type\":\"foundation.two_phase_fluid.two_phase_fluid\"},{\"id\":\"L\",\"label\":\"L\",\"type\":\"output\"}],\"Top\":[]}"
  Steam Generator : SimscapeFluids_lib/Fluid Network Interfaces/Heat Exchangers/Condenser Evaporator (TL-2P)  flow_arrangement=fluids.interfaces.heat_exchangers.enum.FlowArrangementTL2P.Cross  cross_flow_arrangement=fluids.interfaces.heat_exchangers.enum.CrossFlowArrangementTL2P.MixedUnmixed  R_wall=0 K/kW  area_A1=4.56E-3 m^2  area_B1=4.56E-3 m^2  area_A2=2.03e-3 m^2  area_B2=4.03e-3 m^2  flow_geometry_TL=fluids.interfaces.heat_exchangers.enum.FlowGeometryTL.AcrossTubeBank  tube_num_TL=25  tube_length_TL=1 m  tube_cross_section_TL=fluids.interfaces.heat_exchangers.enum.TubeCrossSection.Circular  tube_diameter_TL=0.05 m  tube_width_TL=0.05 m  tube_height_TL=0.05 m  tube_inner_diameter_TL=0.05 m  tube_outer_diameter_TL=0.1 m  tube_flow_area_TL=0.002 m^2  tube_wetted_perimeter_TL=0.15 m  tube_heat_perimeter_TL=0.15 m  tube_pressure_loss_spec_TL=fluids.interfaces.heat_exchangers.enum.TubePressureLossSpec.Haaland  tube_loss_coeff_TL=10  tube_length_add_TL=0.1 m  tube_roughness_pressure_TL=15e-6 m  tube_Re_lam_pressure_TL=2000  tube_Re_tur_pressure_TL=4000  tube_shape_factor_generic_TL=64  tube_heat_coeff_spec_TL=fluids.interfaces.heat_exchangers.enum.TubeHeatCoeffSpec.Gneilinski  tube_colburn_coeff_TL=[.023, .8, .33]  tube_roughness_heat_TL=15e-6 m  tube_Re_lam_heat_TL=2000  tube_Re_tur_heat_TL=4000  tube_Nu_lam_generic_TL=3.66  bank_arrangement_TL=fluids.interfaces.heat_exchangers.enum.BankArrangement.Staggered  bank_num_rows_TL=14  bank_tubes_per_row_TL=12  bank_width_TL=5 m  bank_tube_diameter_TL=0.018 m  bank_longitudinal_pitch_TL=0.03 m  bank_transverse_pitch_TL=0.03 m  bank_pressure_loss_spec_TL=fluids.interfaces.heat_exchangers.enum.BankPressureLossSpec.Martin  bank_euler_TL=10  bank_heat_coeff_spec_TL=fluids.interfaces.heat_exchangers.enum.BankHeatCoeffSpec.Martin  bank_colburn_coeff_TL=[.27, .63, .36]  generic_flow_area_TL=0.01 m^2  generic_heat_area_TL=2 m^2  generic_volume_TL=0.05 m^3  generic_loss_coeff_TL=10  generic_colburn_coeff_TL=[.023, .8, .33]  fouling_factor_TL=0 K*m^2/kW  fin_area_TL=0 m^2  fin_efficiency_TL=0.5  p_init_TL=15 MPa  T_init_TL=300 degC  tube_num_2P=370  tube_length_2P=10 m  tube_cross_section_2P=fluids.interfaces.heat_exchangers.enum.TubeCrossSection.Circular  tube_diameter_2P=0.025 m  tube_width_2P=0.05 m  tube_height_2P=0.05 m  tube_inner_diameter_2P=0.05 m  tube_outer_diameter_2P=0.1 m  tube_flow_area_2P=0.002 m^2  tube_wetted_perimeter_2P=0.15 m  tube_heat_perimeter_2P=0.15 m  tube_pressure_loss_spec_2P=fluids.interfaces.heat_exchangers.enum.TubePressureLossSpec2P.Haaland  tube_loss_coeff_2P=10  tube_length_add_2P=0.4 m  tube_roughness_pressure_2P=15e-6 m  tube_Re_lam_pressure_2P=2000  tube_Re_tur_pressure_2P=4000  tube_shape_factor_generic_2P=64  tube_heat_coeff_spec_2P=fluids.interfaces.heat_exchangers.enum.TubeHeatCoeffSpec2P.GneilinskiCavalliniZecchin  tube_colburn_coeff_liq_2P=[.023, .8, .33]  tube_colburn_coeff_mix_2P=[.05, .8, .33]  tube_colburn_coeff_vap_2P=[.023, .8, .33]  tube_roughness_heat_2P=15e-6 m  tube_Re_lam_heat_2P=2000  tube_Re_tur_heat_2P=4000  tube_Nu_lam_generic_2P=3.66  fouling_factor_2P=0 K*m^2/kW  fin_area_2P=0 m^2  fin_efficiency_2P=0.5  energy_spec_2P=foundation.enum.energy_spec.temperature  p_init_2P=4 MPa  T_init_2P=225 degC  x_init_2P=0.5  alpha_init_2P=0.5  h_init_2P=483 kJ/kg  u_init_2P=1500 kJ/kg
      settings: InternalSimscapePortConfiguration="{\"Bottom\":[],\"Left\":[{\"id\":\"A1\",\"label\":\"A1\",\"type\":\"foundation.thermal_liquid.thermal_liquid\"},{\"id\":\"B1\",\"label\":\"B1\",\"type\":\"foundation.thermal_liquid.thermal_liquid\"}],\"Right\":[{\"id\":\"A2\",\"label\":\"A2\",\"type\":\"foundation.two_phase_fluid.two_phase_fluid\"},{\"id\":\"B2\",\"label\":\"B2\",\"type\":\"foundation.two_phase_fluid.two_phase_fluid\"}],\"Top\":[{\"id\":\"Z\",\"label\":\"Z\",\"type\":\"output\"}]}"
  Step : Step  Time=7  After=800  SampleTime=0
  Step1 : Step  Time=17  After=-800  SampleTime=0
  Subsystem : Subsystem
  Subsystem1 : Subsystem
  Subtract : Sum
  Subtract1 : Sum  Inputs=+-
  Subtract2 : Sum  Inputs=+-
  Subtract3 : Sum  Inputs=+-
  Subtract4 : Sum  Inputs=-+
  Switch : Switch  Threshold=3600  SaturateOnIntegerOverflow=off  InputSameDT=off
  Switch1 : Switch  Threshold=0.5  SaturateOnIntegerOverflow=off  InputSameDT=off
  Synchronous Machine Measurement : ee_lib/Electromechanical/Synchronous/Synchronous Machine Measurement  output_idx=3
      settings: InternalSimscapePortConfiguration="{\"Bottom\":[],\"Left\":[{\"id\":\"pu_input\",\"label\":\"pu\",\"type\":\"input\"}],\"Right\":[{\"id\":\"pu_output\",\"label\":\"o\",\"type\":\"output\"}],\"Top\":[]}"
  Synchronous Machine Round Rotor : ee_lib/Electromechanical/Synchronous/Synchronous Machine Round Rotor  port_option=ee.enum.threePhasePort.composite  SRated=15E6 A*V  VRated=24e3 V  FRated=60 Hz  nPolePairs=1  param_option=ee.enum.sm.parameterization.fundamental  fieldCircuitParameterization_option=ee.enum.sm.fieldparameterization.current  baseEfd=92.95 V  baseIfd=1300 A  zero_sequence=ee.enum.park.zerosequence.exclude  axes_param=ee.enum.rotorangle.daxis  Ladu=1.66  Laqu=1.61  L0=0.15  Ll=0.15  Ra=0.003  Lfd=0.165  Rfd=0.0006  L1d=0.1713  R1d=0.0284  L1q=0.7252  R1q=0.00619  L2q=0.125  R2q=0.02368  Xl=0.15  Xd=1.81  Xq=1.76  X0=0.15  Xdd=0.3  Xqd=0.65  Xddd=0.23  Xqdd=0.25  d_option=ee.enum.circuit.open  Td0d=8 s  Tdd=1.3260 s  Td0dd=0.03 s  Tddd=0.0230 s  q_option=ee.enum.circuit.open  Tq0d=1 s  Tqd=0.3693 s  Tq0dd=0.07 s  Tqdd=0.0269 s  saturation_option=ee.enum.saturation.exclude  saturation_ifd=[0, .48, .76, 1.38, 1.79]  saturation_Vag=[0, .8, 1.08, 1.31, 1.4]  initialization_option=ee.enum.sm.initialization.electrical  source_type=ee.enum.sm.load_flow_source_type.Swing  Vmag0=24e3 V  Vang0=0 deg  Pt0=100e3 A*V  Qt0=0 A*V  minimum_pu=0.95  phase_search_range=[-inf, inf] deg  gmin=1e-6 S  connection_option=ee.enum.Connection.wye  num_q_dampers=2  rotor_offset=-pi / 2 rad  pu_psid_specify=off  pu_psid_priority=None  pu_psid=0  pu_psid_nominal_specify=off  pu_psid_nominal_unit=1  pu_psid_nominal_value=1  pu_psiq_specify=off  pu_psiq_priority=None  pu_psiq=0  pu_psiq_nominal_specify=off  pu_psiq_nominal_unit=1  pu_psiq_nominal_value=1  pu_psifd_specify=off  pu_psifd_priority=None  pu_psifd=0  pu_psifd_nominal_specify=off  pu_psifd_nominal_unit=1  pu_psifd_nominal_value=1  pu_psi1d_specify=off  pu_psi1d_priority=None  pu_psi1d=0  pu_psi1d_nominal_specify=off  pu_psi1d_nominal_unit=1  pu_psi1d_nominal_value=1  pu_psi1q_specify=off  pu_psi1q_priority=None  pu_psi1q=0  pu_psi1q_nominal_specify=off  pu_psi1q_nominal_unit=1  pu_psi1q_nominal_value=1  pu_psi2q_specify=off  pu_psi2q_priority=None  pu_psi2q=0  pu_psi2q_nominal_specify=off  pu_psi2q_nominal_unit=1  pu_psi2q_nominal_value=1  angular_position_diff_specify=off  angular_position_diff_priority=None  angular_position_diff=180 deg  angular_position_diff_nominal_specify=off  angular_position_diff_nominal_unit=deg  angular_position_diff_nominal_value=1  Tmeas=298.15 K  alpha=3.93e-3 1/K  stator_thermal_mass=100 J/K  rotor_thermal_mass=200 J/K  temperatureA_specify=off  temperatureA_priority=High  temperatureA=25 degC  temperatureA_nominal_specify=off  temperatureA_nominal_unit=degC  temperatureA_nominal_value=1  temperatureB_specify=off  temperatureB_priority=High  temperatureB=25 degC  temperatureB_nominal_specify=off  temperatureB_nominal_unit=degC  temperatureB_nominal_value=1  temperatureC_specify=off  temperatureC_priority=High  temperatureC=25 degC  temperatureC_nominal_specify=off  temperatureC_nominal_unit=degC  temperatureC_nominal_value=1  temperatureR_specify=off  temperatureR_priority=High  temperatureR=25 degC  temperatureR_nominal_specify=off  temperatureR_nominal_unit=degC  temperatureR_nominal_value=1
      settings: InternalSimscapePortConfiguration="{\"Bottom\":[],\"Left\":[{\"id\":\"fd_p\",\"label\":\"fd+\",\"type\":\"foundation.electrical.electrical\"},{\"id\":\"fd_n\",\"label\":\"fd-\",\"type\":\"foundation.electrical.electrical\"},{\"id\":\"R\",\"label\":\"R\",\"type\":\"foundation.mechanical.rotational.rotational\"},{\"id\":\"C\",\"label\":\"C\",\"type\":\"foundation.mechanical.rotational.rotational\"}],\"Right\":[{\"id\":\"pu_output\",\"label\":\"pu\",\"type\":\"output\"},{\"id\":\"N\",\"label\":\"~\",\"type\":\"foundation.electrical.three_phase\"}],\"Top\":[]}"
  Tank (G-TL)1 : SimscapeFluids_lib/Fluid Network Interfaces/Tanks & Accumulators/Tank (G-TL)  volume_total=1 m^3  volume_spec=fluids.interfaces.tanks_accumulators.enum.VolumeSpec.Constant  tank_area=0.5 m^2  level_TLU=[0, 3, 5] m  volume_TLU=[0, 4, 6] m^3  inlet_height=0.1 m  inlet_areas_A1B1=[.01, .01] m^2  area_A2=0.01 m^2  g=9.81 m/s^2  p_gas_tank_specify=on  p_gas_tank_priority=High  p_gas_tank=15 MPa  p_gas_tank_nominal_specify=off  p_gas_tank_nominal_unit=MPa  p_gas_tank_nominal_value=1  T_gas_tank_specify=on  T_gas_tank_priority=High  T_gas_tank=315 degC  T_gas_tank_nominal_specify=off  T_gas_tank_nominal_unit=K  T_gas_tank_nominal_value=1  rho_gas_tank_specify=off  rho_gas_tank_priority=None  rho_gas_tank=1.2 kg/m^3  rho_gas_tank_nominal_specify=off  rho_gas_tank_nominal_unit=kg/m^3  rho_gas_tank_nominal_value=1  T_liquid_tank_specify=on  T_liquid_tank_priority=High  T_liquid_tank=315 degC  T_liquid_tank_nominal_specify=off  T_liquid_tank_nominal_unit=K  T_liquid_tank_nominal_value=1  level_specify=on  level_priority=High  level=1 m  level_nominal_specify=off  level_nominal_unit=m  level_nominal_value=1  volume_liquid_specify=off  volume_liquid_priority=None  volume_liquid=5 m^3  volume_liquid_nominal_specify=off  volume_liquid_nominal_unit=m^3  volume_liquid_nominal_value=1  mass_liquid_specify=off  mass_liquid_priority=None  mass_liquid=5000 kg  mass_liquid_nominal_specify=off  mass_liquid_nominal_unit=kg  mass_liquid_nominal_value=1  inlet_heights_A2B2=[.1, .1] m  inlet_areas_A2B2=[.01, .01] m^2  inlet_heights_A2B2C2=[.1, .1, .1] m  inlet_areas_A2B2C2=[.01, .01, .01] m^2
      settings: InternalSimscapePortConfiguration="{\"Bottom\":[],\"Left\":[{\"id\":\"A1\",\"label\":\"A1\",\"type\":\"foundation.gas.gas\"},{\"id\":\"B1\",\"label\":\"B1\",\"type\":\"foundation.gas.gas\"},{\"id\":\"A2\",\"label\":\"A2\",\"type\":\"foundation.thermal_liquid.thermal_liquid\"}],\"Right\":[{\"id\":\"H1\",\"label\":\"H1\",\"type\":\"foundation.thermal.thermal\"},{\"id\":\"H2\",\"label\":\"H2\",\"type\":\"foundation.thermal.thermal\"},{\"id\":\"V_out\",\"label\":\"V\",\"type\":\"output\"},{\"id\":\"L_out\",\"label\":\"L\",\"type\":\"output\"}],\"Top\":[]}"
  Thermal Liquid Properties (TL) : SimscapeFluids_lib/Thermal Liquid/Utilities/Thermal Liquid Properties (TL)  fluid_list=fluids.thermal_liquid.utilities.enum.thermal_liquid_fluid_list.water  concentration_param_EG=fluids.thermal_liquid.utilities.enum.thermal_liquid_concentration.volume_fraction  concentration_param_PG=fluids.thermal_liquid.utilities.enum.thermal_liquid_concentration.volume_fraction  c_mass_SW=3.5e-3  c_mass_EG=0.1  c_mass_PG=0.1  c_mass_GL=0.1  c_vol_EG=0.1  c_vol_PG=0.1  beta_const_EG=2.1791 GPa  beta_const_PG=2.1791 GPa  beta_const_GL=2.1791 GPa  p_min_EG=0.01 MPa  p_min_PG=0.01 MPa  p_min_GL=0.01 MPa  p_max_EG=50 MPa  p_max_PG=50 MPa  p_max_GL=50 MPa  p_atm=0.101325 MPa
  Thermal Liquid Properties (TL)1 : SimscapeFluids_lib/Thermal Liquid/Utilities/Thermal Liquid Properties (TL)  fluid_list=fluids.thermal_liquid.utilities.enum.thermal_liquid_fluid_list.water  concentration_param_EG=fluids.thermal_liquid.utilities.enum.thermal_liquid_concentration.volume_fraction  concentration_param_PG=fluids.thermal_liquid.utilities.enum.thermal_liquid_concentration.volume_fraction  c_mass_SW=3.5e-3  c_mass_EG=0.1  c_mass_PG=0.1  c_mass_GL=0.1  c_vol_EG=0.1  c_vol_PG=0.1  beta_const_EG=2.1791 GPa  beta_const_PG=2.1791 GPa  beta_const_GL=2.1791 GPa  p_min_EG=0.01 MPa  p_min_PG=0.01 MPa  p_min_GL=0.01 MPa  p_max_EG=50 MPa  p_max_PG=50 MPa  p_max_GL=50 MPa  p_atm=0.101325 MPa
  Thermal Reference : fl_lib/Thermal/Thermal Elements/Thermal Reference
  Thermodynamic Properties Sensor (2P){,1..4} (5 alike) : fl_lib/Two-Phase Fluid/Sensors/Thermodynamic Properties Sensor (2P)
      settings: InternalSimscapePortConfiguration="{\"Bottom\":[],\"Left\":[{\"id\":\"A\",\"label\":\"A\",\"type\":\"foundation.two_phase_fluid.two_phase_fluid\"}],\"Right\":[{\"id\":\"T\",\"label\":\"T\",\"type\":\"output\"},{\"id\":\"H\",\"label\":\"h\",\"type\":\"output\"},{\"id\":\"V\",\"label\":\"v\",\"type\":\"output\"},{\"id\":\"S\",\"label\":\"s\",\"type\":\"output\"}],\"Top\":[]}"
  Two-Phase Fluid Properties (2P) : fl_lib/Two-Phase Fluid/Utilities/Two-Phase Fluid Properties (2P)  u_min=0 kJ/kg  u_max=4000 kJ/kg  p_TLU=[.001; .00112274217372259; .00126054998865532; .00141527263434886; .00158898627389893; .00178402190317264; .00200299662953676; .00224884878980512; .00252487737863921; .00283478631647638; .00318273415099974; .00357338985907456; .00401199549793563; .00450443654631748; .00505732087940796; .00567806743735912; .00637500577716403; .00715748784374719; .00803601346008173; .00902237122023614; .01012979667594; .0113731499393128; .0127691150849369; .014336424026976; .0160961078754557; .0180717791445625; .0202899485998006; .0227803809956597; .0255764944772957; .0287158090056427; .032240449823198; .0361977127162914; .0406406986588747; .0456290263538697; .0512296322333889; .0575176686527238; .0645775123306147; .0725038965676716; .0814031824357453; .091394785995845; .102612780695886; .115207696450218; .12934853954209; .145225060453328; .163050300052364; .183063448306911; .205533053881254; .230760627686481; .259084688738309; .290885306612289; .326589201449842; .36667546995012; .411682014182549; .462212759485809; .518945758307413; .582642288726182; .654157069747138; .734449730443899; .824597686848553; .925810599378961; 1.03944660480215; 1.16703054054413; 1.31027440589116; 1.47110033464331; 1.65166638748146; 1.85439551014547; 2.08200804600213; 2.33755823927635; 2.62447521876828; 2.94660901200096; 3.30828220724452; 3.71434795664948; 4.17025509881069; 4.68212127461642; 5.25681501749562; 5.90204791960057; 6.62647811066722; 7.43982643809567; 8.35300690722631; 9.37827313213906; 10.529382762142; 11.8217820903244; 13.2728133213656; 14.9019472798441; 16.7310446816716; 18.7846494745497; 21.0903181836728; 23.6789896820378; 26.5854003471659; 29.8485501750623; 33.5122261060171; 37.6255895845526; 42.2438362377545; 47.4289365239576; 53.2504672902587; 59.7865453972087; 67.1248759386262; 75.3639291221923; 84.6142616029251; 95] MPa  p_crit=22.0640 MPa  critical_region=foundation.enum.critical_region.clip  p_crit_fraction=0.12  p_atm=0.101325 MPa  q_rev=0.01 Pa  unorm_liq=[-1; -.958333333333333; -.916666666666667; -.875; -.833333333333333; -.791666666666667; -.75; -.708333333333333; -.666666666666667; -.625; -.583333333333333; -.541666666666667; -.5; -.458333333333333; -.416666666666667; -.375; -.333333333333333; -.291666666666667; -.25; -.208333333333333; -.166666666666667; -.125; -.0833333333333334; -.0416666666666666; 0]  v_liq=[.00100020732544948, .00100020726300335, .0010002071928919, .00100020711417503, .00100020702579618, .00100020692656954, .00100020681516375, .00100020669008383, .00100020654965104, .00100020639198192, .00100020621496035, .00100020601621096, .0010002057930668, .00100020554253399, .00100020526125081, .00100020494544269, .00100020459087245, .00100020419278253, .00100020374583102, .00100020324402174, .00100020268062136, .00100020204807013, .00100020133788097, .00100020054052585, .00100019964530644, .00100019864021207, .00100019751175783, .00100019624480464, .00100019482234984, .00100019322532132, .00100019143228968, .00100018941920187, .00100018715905485, .0010001846215314, .00100018177259635, .00100017857403912, .00100017498296268, .00100017095120895, .00100016642471372, .00100016134278426, .00100015563728587, .00100014923173247, .00100014204026295, .0010001339664942, .00100012490223458, .00100011472603939, .00100010330159183, .00100009047588614, .00100007607718989, .00100005991276002, .00100004176628202, .00100002139499759, .000999998526488461, .000999972855070674, .000999944037755854, .000999911689729031, .000999875379285172, .000999834622163514, .000999788875208073, .000999737529277352, .000999679901338164, .000999615225595999, .000999542643635775, .000999461193403645, .000999369796933885, .000999267246682345, .000999152190329382, .000999023113898678, .000998878323031051, .000998715922248806, .000998533792028207, .000998329563528631, .00099810059074289, .000997843919977287, .00099755625644641, .000997233927872258, .000996872844988745, .000996468458927233, .000996015715464286, .000995509006340398, .000994942117859915, .000994308177257196, .000993599597452603, .000992808021236635, .000991924266119846, .000990938271667886, .000989839049486992, .00098861465356352, .000987252130433194, .00098573752739359, .000984055890597038, .000982191303665813, .000980126959459537, .000977845275147052, .000975328058847084, .000972556735510835, .000969512637773578, .000966177363700338, .000962533197025544, .000958563576309327; .00100018841892372, .00100018398406645, .00100017957534042, .00100017519359941, .00100017083972868, .00100016651463355, .00100016221922754, .00100015795441909, .00100015372109739, .00100014952011441, .0010001453522674, .00100014121827947, .00100013711877363, .00100013305424789, .00100012902504422, .00100012503131558, .00100012107298655, .00100011714970979, .00100011326081664, .00100010940526175, .00100010558155903, .00100010178770971, .00100009802112334, .0010000942785241, .00100009055585109, .00100008684813776, .00100008314938399, .00100007945240635, .00100007574866693, .00100007202810543, .00100006827889624, .0010000644872314, .001000060637045, .00100005670971236, .00100005268370909, .00100004853422766, .00100004423274798, .00100003974655211, .00100003503818065, .00100003006482113, .00100002477762103, .00100001912091604, .00100001303136393, .00100000643697221, .0009999992560071, .000999991395769273, .000999982751221926, .000999973203452171, .000999962617946626, .000999950842660616, .000999937705855753, .000999923013680387, .000999906547461252, .0009998880606778, .000999867275578685, .000999843879404625, .000999817520172301, .000999787801972537, .000999754279728057, .000999716453375443, .000999673761357246, .000999625573433289, .000999571182686054, .000999509796671866, .000999440527639205, .000999362381740551, .000999274247163053, .000999174881113644, .000999062895600234, .000998936741974201, .000998794694225883, .000998634831102159, .000998455017117626, .000998252882786181, .000998025804468552, .000997770884629068, .000997484933794632, .000997164456428082, .000996805644437897, .000996404385103752, .000995956296002551, .000995456813315116, .000994901398520536, .000994286064982048, .000993608978406738, .000992876136881603, .000992129193475016, .000991517986232412, .000990372765199316, .000989072075354225, .000987603993568335, .000985974124940594, .000984176896118864, .00098218367245538, .00097997283525223, ...(+45851 chars)] m^3/kg  s_liq=[-7.05045840376749e-13, -7.87027914839162e-13, -1.21661398502221e-12, -1.55110084882885e-12, -1.94461480624843e-12, -2.57423713811976e-12, -3.47767959869555e-12, -4.23355432523899e-12, -5.633808157057e-12, -6.99471059313305e-12, -8.95900109725246e-12, -1.16644095545121e-11, -1.46190435181374e-11, -1.85181109795698e-11, -2.34419543717823e-11, -2.9602087446888e-11, -3.75576279527205e-11, -4.73397290775756e-11, -5.97059051894859e-11, -7.54989320139251e-11, -9.51106838668235e-11, -1.20025036295951e-10, -1.50382998469382e-10, -1.91083819156992e-10, -2.4088301046844e-10, -3.03792775127917e-10, -3.82934990530951e-10, -4.82864580734676e-10, -6.08756254279156e-10, -7.67524379324554e-10, -9.67604911333051e-10, -1.21979652915284e-09, -1.53762135614574e-09, -1.93831202436376e-09, -2.44343309867349e-09, -3.08014851962731e-09, -3.88256610948456e-09, -4.89435771931136e-09, -6.16946263517951e-09, -7.77685893490021e-09, -9.80304590523874e-09, -1.23568744257418e-08, -1.55761776789201e-08, -1.96341969052447e-08, -2.47486404223749e-08, -3.11956976409671e-08, -3.93217706995304e-08, -4.95645881278834e-08, -6.24749022229816e-08, -7.87473126692738e-08, -9.92574683644515e-08, -1.25108228246296e-07, -1.57689670531543e-07, -1.98753937430942e-07, -2.50508563542826e-07, -3.15734782545124e-07, -3.97937631454781e-07, -5.01532810730435e-07, -6.32083273061825e-07, -7.96597406931389e-07, -1.00390280108994e-06, -1.2651187351257e-06, -1.59424877541207e-06, -2.00892781216652e-06, -2.53136011638268e-06, -3.18950035883824e-06, -4.01853639364152e-06, -5.06275397494756e-06, -6.37787768131054e-06, -8.03401011078313e-06, -1.01193201823024e-05, -1.274466856761e-05, -1.60494023777535e-05, -2.02086165351325e-05, -2.54422366036015e-05, -3.20263747503063e-05, -4.03075125675031e-05, -5.07201925779572e-05, -6.38090591041844e-05, -8.02562733315751e-05, -.000100915557822456, -.000126854393027582, -.000159406201949221, -.000200234726866816, -.000251413225381822, -.000315521587717782, -.000395765133786477, -.000496118152201492, -.000621500275714703, -.000777985262661619, -.000973053511344264, -.00121589078170344, -.0015177400674783, -.00189231176510098, -.00235625635801383, -.00292970204819937, -.00363685724598224, -.00450667471591771, -.00557357093569877, -.00687819175416438; .00446657256953546, .00555283262208184, .00665298270232147, .00776741393348658, .00889652271648415, .0100407115885335, .0112003900263792, .0123759752213135, .0135678928259572, .0147765776883396, .0160024745935744, .0172460389988151, .0185077377960502, .0197880500877376, .0210874679887233, .0224064974657629, .0237456592090053, .0251054895494021, .0264865414159024, .0278893853519512, .0293146105749496, .0307628261060538, .0322346619545676, .0337307703721922, .0352518271800654, .0367985331682527, .0383716155815334, .0399718296890423, .0415999604467728, .0432568242596421, .0449432708491413, .0466601852347832, .0484084898364029, .0501891467098943, .0520031599194747, .0538515780731902, .0557354970052083, .0576560626600314, .0596144741562925, .0616119870712367, .0636499169574331, .0657296431198309, .0678526126673146, .0700203448897714, .0722344359697157, .0744965640855095, .0768084949402807, .0791720877711655, .0815893018939807, .0840622038524436, .0865929752465348, .0891839213348152, .0918374805045949, .0945562347480557, .0973429212749736, .100200445439143, .103131895184885, .106140557252666, .10922993544547, .112403771311118, .115666067692799, .119021115681489, .122473525670754, .126028263375389, .129690691918979, .133466621426034, .13736236799356, .14138482453151, .145541546837596, .149840859512912, .154291988152232, .158905226949536, .163692154956815, .168665920558703, .173841623753384, .179236842022868, .184872372533219, .190773309657136, .196970659381392, .203503848522254, .210424811318855, .217805120343344, .225749966246503, .234431267808216, .244186002630389, .25585506253651, .272386089674436, .302100195471736, .306557382400805, .309819708675095, .312056289947511, .314369304579656, .317236085935913, ...(+41434 chars)] kJ/(K*kg)  T_liq=[273.159998291077, 273.159997751012, 273.159997144593, 273.159996463772, 273.159995699381, 273.159994841165, 273.159993877586, 273.159992795785, 273.159991581167, 273.159990217533, 273.15998868659, 273.159986967561, 273.159985037678, 273.159982870932, 273.159980438272, 273.159977707056, 273.159974640676, 273.159971197971, 273.159967332851, 273.159962993325, 273.15995812136, 273.159952651571, 273.15994651064, 273.159939616193, 273.159931875935, 273.159923186012, 273.159913430085, 273.159902477298, 273.159890181062, 273.159876376717, 273.159860879444, 273.159843481712, 273.159823950889, 273.159802025583, 273.159777412762, 273.15974978335, 273.159718768375, 273.159683953724, 273.15964487493, 273.15960101081, 273.159551777112, 273.159496518496, 273.159434500105, 273.159364898222, 273.159286789452, 273.159199139166, 273.159100788117, 273.158990437735, 273.158866634217, 273.158727750094, 273.158571964373, 273.158397240334, 273.158201301104, 273.157981602771, 273.157735304847, 273.157459237733, 273.157149867811, 273.156803258854, 273.156415030765, 273.15598031553, 273.155493710064, 273.154949226642, 273.154340241463, 273.15365944232, 273.15289877633, 273.152049399179, 273.151101629486, 273.150044909347, 273.148867777435, 273.147557858815, 273.146101879204, 273.144485713376, 273.142694478879, 273.140712692165, 273.138524505606, 273.136114050981, 273.133465921939, 273.130565834149, 273.127401513117, 273.123963872893, 273.120248560551, 273.116257960298, 273.112003772616, 273.107510304394, 273.102818635673, 273.09799185537, 273.093121581246, 273.088336079303, 273.083810074793, 273.079776855107, 273.076542641094, 273.074503655632, 273.074165978154, 273.076168166967, 273.081306335056, 273.09056091525, 273.105123705308, 273.126422900983, 273.156142700744, 273.196232754335; 273.449312358855, 273.519728944504, 273.59106844902, 273.663357090888, 273.736621473863, 273.810888644354, 273.886186145644, 273.962542069657, 274.039985107551, 274.118544600161, 274.198250587757, 274.279133861214, 274.361226013826, 274.44455949466, 274.52916766458, 274.6150848534, 274.702346421062, 274.790988820835, 274.881049666415, 274.972567802078, 275.065583377749, 275.160137927054, 275.256274451108, 275.354037506327, 275.453473298113, 275.554629779724, 275.657556757525, 275.762306002249, 275.86893136765, 275.977488916404, 276.088037053727, 276.200636670347, 276.315351293762, 276.432247250566, 276.551393839299, 276.672863514847, 276.7967320868, 276.923078930748, 277.051987216416, 277.1835441519, 277.317841247356, 277.45497459922, 277.595045198099, 277.73815926159, 277.884428596155, 278.033970991383, 278.186910649497, 278.343378655705, 278.503513493927, 278.66746161399, 278.835378057316, 279.007427148686, 279.18378326455, 279.364631687036, 279.550169558546, 279.740606951193, 279.936168069282, 280.137092606683, 280.343637286029, 280.556077609996, 280.774709864503, 280.999853420766, 281.231853395056, 281.471083739539, 281.717950857139, 281.972897858885, 282.236409616944, 282.509018813934, 282.791313255902, 283.083944810539, 283.387640467934, 283.703216222701, 284.031594776823, 284.373828526496, 284.7311300231, 285.104913274297, 285.496851198425, 285.908957876567, 286.343710196733, 286.80423471511, 287.294608837676, 287.82038143902, 288.389584213715, 289.015106184942, 289.721704208206, 290.57014624382, 291.771628182453, 293.926669322509, 294.296938773523, 294.590451085784, 294.819945413856, 295.065883053589, 295.364648699239, 295.670908060714, 295.970789164316, 296.251012375539, 296.497195783816, 296.697915573608, 296.853023135695, 296.982558622146; 273.738693844061, 273.879563825998, 274.022287862787, 274.166918593293, 274.31350943525, 274.462114700155, 274.612789701487, 274.76559085912, 274.92057580033, 275.077803460773, 275.237334184965, 275.399229828111, 275.563553860703, 275.730371475718, 275.899749700306, 276.071757511918, 276.246465959942, 276.423948293574, 276.604280096033, 276.787539426652, 276.973806970093, 277.163166195266, 277.35570352231, 277.551508500318, ...(+40704 chars)] K  nu_liq=[1.7917284815762, 1.79172812803551, 1.79172773110138, 1.79172728544635, 1.7917267850908, 1.79172622332123, 1.7917255926019, 1.7917248844648, 1.79172408941084, 1.79172319677148, 1.79172219456638, 1.79172106936268, 1.79171980604367, 1.79171838766791, 1.79171679520303, 1.79171500728093, 1.79171299991296, 1.79171074616787, 1.79170821579955, 1.79170537487376, 1.79170218526332, 1.79169860417681, 1.79169458356931, 1.79169006950841, 1.79168500142722, 1.79167931134595, 1.79167292292763, 1.79166575048946, 1.7916576977831, 1.79164865686523, 1.79163850644601, 1.79162711040036, 1.79161431589773, 1.79159995137726, 1.79158382423148, 1.79156571825254, 1.79154539071544, 1.79152256915611, 1.79149694771436, 1.79146818307401, 1.79143588984344, 1.79139963545289, 1.79135893437743, 1.79131324166523, 1.79126194570662, 1.79120436008817, 1.79113971450312, 1.79106714454662, 1.79098568025457, 1.79089423332076, 1.7907915827457, 1.79067635877515, 1.79054702494118, 1.79040185796044, 1.79023892526431, 1.79005605990856, 1.78985083251562, 1.78962052001425, 1.78936207075003, 1.78907206559537, 1.78874667480049, 1.78838160978626, 1.78797206988038, 1.78751268313864, 1.78699744091201, 1.7864196256097, 1.7857717310849, 1.78504537525806, 1.78423120438025, 1.78331878866103, 1.78229650891305, 1.78115143425944, 1.77986919075408, 1.77843382179501, 1.77682764101537, 1.7750310793466, 1.77302252860231, 1.77077818526512, 1.76827189907313, 1.76547503351357, 1.76235634703284, 1.758881907221, 1.75501505335383, 1.75071642824654, 1.745944104972, 1.74065384192818, 1.7347994963663, 1.72833372601204, 1.72120880692642, 1.71337803363744, 1.70479739947197, 1.69542789316032, 1.68523844626116, 1.67420966196635, 1.66233844301517, 1.64964362261559, 1.63617267029781, 1.6220094907655, 1.6072832556805, 1.59217811011515; 1.77377767764156, 1.76945208477402, 1.76508707935446, 1.7606816425659, 1.75623475962728, 1.75174541707923, 1.74721260035302, 1.74263529157421, 1.73801246752514, 1.73334309768936, 1.72862614243819, 1.72386055122211, 1.71904526079301, 1.71417919345131, 1.70926125521941, 1.70429033406154, 1.69926529796561, 1.69418499302564, 1.6890482414172, 1.68385383932616, 1.67860055472268, 1.6732871251083, 1.66791225510158, 1.66247461393328, 1.65697283281412, 1.6514055021531, 1.64577116865579, 1.64006833226969, 1.63429544293076, 1.62845089727558, 1.62253303492034, 1.61654013477715, 1.61047041106622, 1.60432200909119, 1.59809300077834, 1.59178137996637, 1.58538505736123, 1.57890185522567, 1.57232950166204, 1.56566562455975, 1.55890774509036, 1.55205327075226, 1.54509948787506, 1.53804355359162, 1.53088248715791, 1.52361316055255, 1.51623228833336, 1.50873641659921, 1.50112191099034, 1.49338494361257, 1.48552147874775, 1.477527257232, 1.46939777927937, 1.46112828566707, 1.45271373695774, 1.44414879057782, 1.43542777545384, 1.4265446638669, 1.41749304007924, 1.40826606539043, 1.39885643878028, 1.38925635272185, 1.37945744304658, 1.36945073181888, 1.35922656173776, 1.34877452016486, 1.33808335024645, 1.32714084573514, 1.31593372480963, 1.30444747634297, 1.29266616930007, 1.28057221182333, 1.26814603997658, 1.25536570654683, 1.24220632413874, 1.22863929133221, 1.214631187907, 1.20014215215067, 1.18512342236084, 1.16951347719231, 1.15323168746793, 1.13616709840039, 1.11815598170334, 1.09892714865166, 1.07793637498657, 1.05380146166027, 1.02169647162528, .969221439548868, .959281874229169, .951067761926794, .9442232584707, .936991769255103, .928644888825034, .920177681459373, .911895500035132, .904078097137958, .89701609509852, .890937051516499, .885861771960224, .881462956503174; 1.75611103161164, 1.74761306951051, 1.7390706786988, 1.73048264698389, 1.72184780313041, 1.71316501180557, 1.70443316922343, 1.69565119929071, 1.68681805023937, 1.67793269150607, 1.6689941109435, 1.6600013122043, 1.65095331223628, 1.64184913894036, 1.63268782885213, 1.62346842489104, 1.61418997413395, 1.604851525575, 1.59545212791799, 1.58599082730083, 1.57646666506041, 1.56687867539715, 1.55722588308673, 1.54750730108287, ...(+40705 chars)] mm^2/s  k_liq=[.5555988310868, .555598923248142, .555599026722272, .555599142896704, .555599273330844, .555599419774665, .555599584192979, .555599768792312, .555599976050098, .555600208746166, .555600470003652, .555600763327632, .555601092654728, .555601462403204, .555601877534417, .555602343618926, .555602866910154, .555603454429339, .555604114060451, .555604854652265, .555605686142374, .5556066196873, .555607667812397, .555608844578954, .55561016577576, .555611649127541, .555613314535305, .55561518434034, .555617283634789, .555619640563828, .555622286751563, .555625257692989, .555628593236699, .555632338120536, .555636542568866, .55564126296576, .555646562610218, .555652512562487, .555659192595951, .555666692261752, .555675112089279, .555684564925419, .555695177444298, .555707091837493, .555720467709421, .555735484206128, .555752342399363, .555771267961732, .555792514167656, .555816365253309, .555843140184561, .555873196880586, .555906936941424, .55594481094515, .555987324378003, .556035044269277, .55608860661666, .556148724685401, .556216198287316, .556291924147729, .556376907449871, .556472274769908, .556579288430578, .556699362514999, .55683408066662, .556985215862944, .557154752345792, .5573449099032, .557558170709648, .557797308921507, .558065423240431, .558365972599454, .558702815227432, .559080251116119, .559503068061265, .559976591258199, .560506736370031, .561100065808182, .561763847884149, .562506118059428, .563335741389024, .564262474700101, .565297026655031, .566451112995284, .5677375036915, .569170057521056, .570763741578253, .572534607349101, .574499778784791, .576677335318942, .579086184262815, .581745844610549, .584676148261707, .587896839774206, .591427059854795, .595284701257021, .599485632919903, .604042800184794, .608965226971595, .614256970135224; .556337890638046, .556517145240949, .556698473970567, .556881934429222, .557067584852239, .557255484255709, .557445692577012, .557638270809519, .557833281135543, .558030787062881, .558230853558009, .558433547184534, .558638936251312, .55884709096173, .559058083576768, .559271988582227, .559488882873482, .559708845949371, .559931960122154, .560158310741455, .560387986440358, .560621079397872, .560857685622523, .561097905264125, .561341842944947, .561589608130291, .561841315520616, .5620970854857, .562357044542232, .562621325838997, .562890069762804, .563163424522684, .563441546831047, .563724602639263, .564012767947248, .564306229691042, .564605186718498, .564909850863169, .565220448127569, .565537219985372, .565860424820472, .566190339514614, .566527261203158, .566871509215378, .567223427222697, .567583385620116, .567951784162428, .568329054890262, .568715665377578, .56911212233625, .569518975622148, .569936822686001, .570366313527763, .570808156202277, .571263122953535, .57173205704266, .572215880355799, .572715601883654, .573232327184098, .573767268914192, .574321758644482, .574897260005425, .57549538342184, .576117902607436, .576766773065013, .577444152874158, .578152426109809, .578894229303079, .579672481469293, .580490418367308, .581351631871181, .582260115610772, .583220318608533, .584237209184366, .585316352719206, .586464008615858, .587687254923603, .588994154365257, .59039398511761, .591897577594168, .593517836443058, .59527061923298, .597176422464569, .599264344018848, .601583834944702, .604244942457816, .607607003893138, .612634941826706, .614800880828557, .617005263125046, .619288627449996, .621798473187162, .624608969154157, .627666554111374, .630969638658207, .634519144180131, .638315614646913, .642364785731255, .64668876436665, .651337292922158; .557072383869131, .557428328848423, .557787845166414, .558151029402328, .558517978479265, .558888789919242, .55926356207716, .559642394363009, .560025387449509, .560412643482964, .560804266281361, .561200361538478, .561601037035101, .56200640284749, .562416571570691, .562831658549019, .563251782117082, .563677063858558, .564107628873501, .56454360607177, .564985128476762, .56543233355755, .565885363574984, ...(+40713 chars)] W/(K*m)  Pr_liq=[13.6057970740934, 13.6057910172678, 13.6057842169634, 13.6057765820043, 13.6057680099124, 13.6057583856797, 13.6057475801822, 13.6057354484133, 13.6057218275651, 13.60570653496, 13.6056893653264, 13.6056700884064, 13.6056484454266, 13.6056241460709, 13.6055968643143, 13.6055662340933, 13.6055318444921, 13.6054932341308, 13.6054498849733, 13.6054012155636, 13.6053465729515, 13.6052852240901, 13.6052163460247, 13.6051390149109, 13.6050521934582, 13.6049547172102, 13.6048452787911, 13.6047224106715, 13.6045844645969, 13.6044295919484, 13.6042557157657, 13.6040605050176, 13.6038413430377, 13.6035952923669, 13.6033190557167, 13.6030089318529, 13.6026607662517, 13.602269895727, 13.6018310862756, 13.6013384635603, 13.6007854346323, 13.6001646006141, 13.5994676584656, 13.5986852910574, 13.5978070440938, 13.5968211881058, 13.5957145641225, 13.5944724108069, 13.5930781710484, 13.5915132758175, 13.5897569024895, 13.5877857047778, 13.585573511438, 13.5830909900135, 13.5803052720266, 13.5771795357155, 13.5736725416529, 13.5697381170314, 13.5653245831502, 13.560374121055, 13.5548220717149, 13.5485961599523, 13.5416156439316, 13.5337903791872, 13.5250197947763, 13.5151917765394, 13.5041814546696, 13.4918498939937, 13.478042687397, 13.4625884567494, 13.4452972684539, 13.4259589795038, 13.4043415289685, 13.3801892117881, 13.353220970219, 13.3231287600369, 13.2895760636566, 13.2521966457231, 13.2105936657372, 13.1643393043767, 13.1129750831427, 13.0560131063686, 12.9929384914732, 12.923213313555, 12.8462824258465, 12.7615815788783, 12.6685481185269, 12.5666359912393, 12.4553318382617, 12.3341788316522, 12.2028024572353, 12.0609422009539, 11.9084879192436, 11.7455207588073, 11.5723578734398, 11.3895996387124, 11.198177435755, 10.9993994380376, 10.7949913081805, 10.5871284907792; 13.4486778700347, 13.4108593388509, 13.3727137727164, 13.3342327371451, 13.2954078507715, 13.2562307616241, 13.2166931258613, 13.1767865884687, 13.1365027653488, 13.0958332262764, 13.0547694787994, 13.013302952547, 12.9714249833524, 12.9291267977354, 12.8863994968977, 12.8432340405694, 12.7996212301233, 12.7555516911928, 12.7110158555266, 12.6660039420621, 12.6205059369579, 12.5745115726281, 12.5280103058583, 12.4809912944004, 12.4334433727374, 12.3853550258218, 12.3367143619693, 12.2875090837468, 12.2377264568962, 12.1873532794604, 12.1363758446623, 12.0847799059452, 12.0325506374205, 11.9796725923615, 11.9261296588559, 11.8719050123814, 11.8169810653521, 11.7613394128016, 11.704960774345, 11.647824931827, 11.5899106622409, 11.531195665502, 11.4716564865855, 11.4112684314494, 11.3500054761353, 11.2878401682822, 11.2247435205253, 11.1606848947224, 11.0956318762097, 11.0295501371659, 10.962403287886, 10.8941527149136, 10.8247574044813, 10.754173750258, 10.6823553432881, 10.6092527427871, 10.5348132255728, 10.4589805119549, 10.3816944652432, 10.3028907632773, 10.2225005348174, 10.1404499613238, 10.0566598350344, 9.97104506816019, 9.8835141441352, 9.79396849945467, 9.70230182039992, 9.60839923333985, 9.51213635817968, 9.41337818177641, 9.31197768797237, 9.2077741522356, 9.1005909578327, 8.99023272431781, 8.87648141439409, 8.75909089807381, 8.63777913209501, 8.51221656586817, 8.38200840206449, 8.24666648240129, 8.10556262752326, 7.95784543917599, 7.80227215150452, 7.63679484002475, 7.45729967398432, 7.25330738443144, 6.98819060922542, 6.56898129606447, 6.47481250055343, 6.39253089256802, 6.3192014196219, 6.24152752473967, 6.15414336966179, 6.06449829911239, 5.9748421772625, 5.88719770186676, 5.80362746395679, 5.72570595588247, 5.65352875798752, 5.58479286703666; 13.2943416367064, 13.2202052139643, 13.1457496655013, 13.0709655915783, 12.9958439951089, 12.9203762367062, 12.8445539957301, 12.7683692360692, 12.6918141759903, 12.6148812604899, 12.5375631366053, 12.4598526301846, 12.3817427237325, 12.3032265357856, 12.2242973005283, 12.1449483479694, 12.0651730844561, 11.9849649730895, 11.9043175144171, 11.8232242265931, 11.7416786258269, 11.6596742061617, 11.5772044194839, ...(+40727 chars)]  u_sat_liq=[29.2976389515495; 36.4274464503909; 43.6502943784891; 50.9688235460151; 58.3857131338879; 65.9036864657328; 73.5255164614608; 81.2540308683062; 89.092117359203; 97.0427285711949; 105.1088871471; 113.293690839202; 121.600317725832; 130.03203157577; 138.592187414229; 147.284237316646; 156.111736468223; 165.078349519158; 174.18785726889; 183.444163708126; 192.851303438662; 202.413449526776; 212.134921787045; 222.020195551149; 232.073910946078; 242.300882717522; 252.706110633902; 263.294790513601; 274.072325914587; 285.044340535623; 296.216691378571; 307.59548272749; 319.1870810067; 330.99813058471; 343.035570598587; 355.306652891555; 367.81896113253; 380.580431257358; 393.599373321438; 406.884494907101; 420.44492623319; 434.290247134865; 448.430516103704; 462.876301606394; 477.638715925801; 492.729451808813; 508.160822239982; 523.945803711925; 540.098083415992; 556.632110843954; 573.563154367692; 590.907363456963; 608.681837305357; 626.904700768179; 645.595188677142; 664.773739795173; 684.462101917128; 704.683449924654; 725.462518980546; 746.825755523466; 768.801489329346; 791.420130682492; 814.714397706377; 838.719580225817; 863.473848283998; 889.018615793402; 915.398973010775; 942.664205969625; 970.868427256292; 1000.07135146045; 1030.33926164708; 1061.74623247584; 1094.37570470146; 1128.32255067815; 1163.69584133093; 1200.62263961127; 1239.25333574224; 1279.76936577674; 1322.39473742031; 1367.41388891791; 1415.20069227449; 1466.26892290803; 1521.37090074044; 1581.73034145221; 1649.73232079058; 1731.30197172385; 1847.17927762085; 2056.34806264226; 2088.50059191893; 2112.4350204755; 2129.37026909632; 2147.13438479139; 2169.16824543376; 2190.91474512801; 2210.90554944606; 2227.7371454335; 2239.91027703293; 2246.22462783334; 2246.56933058969; 2242.74587564859] kJ/kg  unorm_vap=[1; 1.04166666666667; 1.08333333333333; 1.125; 1.16666666666667; 1.20833333333333; 1.25; 1.29166666666667; 1.33333333333333; 1.375; 1.41666666666667; 1.45833333333333; 1.5; 1.54166666666667; 1.58333333333333; 1.625; 1.66666666666667; 1.70833333333333; 1.75; 1.79166666666667; 1.83333333333333; 1.875; 1.91666666666667; 1.95833333333333; 2]  v_vap=[129.178337496409, 115.746508718443, 103.71563820029, 92.9391932584351, 83.2860057998384, 74.638657724233, 66.892036335208, 59.9520418260969, 53.734430801917, 48.1637814930601, 43.1725678315966, 38.7003309160093, 34.6929376015522, 31.1019170368707, 27.883866936451, 24.9999222447121, 22.4152796224809, 20.098771879517, 18.0224870964065, 16.1614277335436, 14.4932055204572, 12.9977683622603, 11.6571558964652, 10.4552806881375, 9.37773236863183, 8.4116023069095, 7.54532665631218, 6.76854584672709, 6.07197879519373, 5.4473102897281, 4.88709016368007, 4.38464302336693, 3.93398742182005, 3.5297634878747, 3.16716812396361, 2.84189697913915, 2.5500924872067, 2.28829733443274, 2.05341278802293, 1.84266137627753, 1.65355346476205, 1.48385732064141, 1.33157230011321, 1.19490483216277, 1.07224690613082, .962156801251009, .863341823764602, .774642841786284, .695020430086296, .623542456638365, .559372960402502, .501762185584318, .450037651730541, .403596151656959, .361896580515287, .324453509426845, .290831426167897, .260639573494369, .233527322941816, .209180028419079, .187315309710778, .16767972118648, .15004576564727, .13420921738119, .119986722198793, .107213645525012, .0957421425748051, .0854394272751407, .0761862189468227, .0678753478476088, .060410502507616, .05370510334634, .0476812883308998, .0422689974063287, .0374051430754911, .0330328547158975, .0291007836853925, .0255624543422632, .0223756415046547, .0195017448151783, .0169051081269986, .0145521786915118, .0124102592355994, .010445171644355, .00861551503536135, .00685243687762084, .00490912079993095, .00317091890440297, .00311263647020915, .0030197960238285, .00290370003970192, .0028016656382173, .00272169001068864, .00264347352918441, .00256249839262667, .00247624386381736, .00238361506529656, .00228538840945448, .00218479924114821, .00208729342673583; 151.21175457965, 135.332534667933, 121.125433141508, 108.413935292645, 97.0402005955536, 86.8630832634907, 77.7563629945979, 69.607163550534, 62.3145391936136, 55.7882111355236, 49.9474380512015, 44.7200064093552, 40.041327887751, 35.8536324965051, 32.1052472433535, 28.7499512563205, 25.74639924567, 23.0576060504072, 20.6504857859626, 18.4954397991009, 16.5659882518001, 14.8384407063007, 13.2916015751581, 11.9065067395572, 10.666188031794, 9.55546262866098, 8.56074471604364, 7.66987706522336, 6.871980411772, 6.15731875172579, 5.51717886970743, 4.94376259241671, 4.43009042065737, 3.96991533585295, 3.55764570462069, 3.18827631903943, 2.85732671220506, 2.56078597980537, 2.29506341990865, 2.05694437598668, 1.84355073329364, 1.65230557692134, 1.48090157188443, 1.32727267210895, 1.18956880679353, 1.06613322980463, .955482251027523, .856287098335552, .767357685439817, .687628084668634, .616143524999628, .552048754722298, .49457762779933, .443043768306104, .396832242390083, .355392074602085, .318229563117309, .284902292779131, .255013774563188, .228208652706057, .204168402842974, .182607492371085, .163269938776807, .145926227526342, .130370555162208, .116418359796932, .103904109921106, .0926793237484216, .082610794355077, .0735789983878082, .0654766683848579, .0582075106996003, .0516850525059235, .045831602345432, .0405773092589148, .0358593058351386, .0316209202438637, .0278109405749205, .0243829098613915, .0212944188695627, .0185063388200109, .0159818776068174, .0136851886509116, .0115787886735364, .00961725306335078, .00772501106492064, .00563001501094613, .00372521425323849, .0036064003602763, .00345676992474126, .00328667110952763, .00313773365071191, .00301824937318557, .00290497425814861, .00279255016052357, .0026780565045257, .00256013081688562, .00243939743909321, .00231904134321985, .00220448022791339; 173.077544485884, 154.770758946119, 138.405023021781, 123.774080450989, 110.693633801704, 98.9990026806603, 88.5430320658742, 79.194224009148, 70.8350688205294, 63.3605544047747, 56.6768347037023, 50.7000402374053, 45.3552155575867, 40.5753700516369, 36.3006299873226, 32.4774809834666, 29.0580912489548, 25.9997069653363, ...(+41655 chars)] m^3/kg  s_vap=[8.97486946817622, 8.93253369462561, 8.89027734151982, 8.84810137095955, 8.80600674459701, 8.76399442129349, 8.72206535459351, 8.68022049000499, 8.63846076207632, 8.59678709125826, 8.55520038053618, 8.51370151181952, 8.47229134206719, 8.43097069912375, 8.38974037724245, 8.34860113225777, 8.30755367636813, 8.26659867248245, 8.22573672806965, 8.18496838845316, 8.14429412946716, 8.10371434939431, 8.06322936008488, 8.02283937714879, 7.98254450910158, 7.9423447453305, 7.90223994273931, 7.86222981092072, 7.82231389569445, 7.78249156084763, 7.74276196790842, 7.70312405378663, 7.66357650611937, 7.62411773617014, 7.58474584914466, 7.54545861180547, 7.50625341729188, 7.46712724707877, 7.42807663003417, 7.38909759856228, 7.35018564183765, 7.31133565614383, 7.27254189232088, 7.23379790028919, 7.19509647054893, 7.15642957243872, 7.11778828877216, 7.07916274623976, 7.04054204066254, 7.00191415580473, 6.96326587398888, 6.92458267620782, 6.88584862879315, 6.84704625297943, 6.80815637290202, 6.76915793668217, 6.73002780428265, 6.69074049474414, 6.65126788420428, 6.61157884469958, 6.57163881205841, 6.53140926906335, 6.49084712727525, 6.44990398715043, 6.40852525087907, 6.36664905502983, 6.32420497958695, 6.2811124749514, 6.23727892733271, 6.1925972537256, 6.14694287702632, 6.10016987258809, 6.05210598562044, 6.00254607231092, 5.95124328607904, 5.89789696757947, 5.84213561343958, 5.78349230480381, 5.7213681741325, 5.6549760200954, 5.58324904786489, 5.50468371073484, 5.41704531414375, 5.31674647840113, 5.19727461928091, 5.04376885853061, 4.79388869527898, 4.47174386166458, 4.51836769363309, 4.55023362733564, 4.56974014168386, 4.59019612523743, 4.61699684652128, 4.64249197878388, 4.66434741984359, 4.68048524717652, 4.68884747851013, 4.68797348716367, 4.67808754343718, 4.66213355191591; 9.26946100074831, 9.22506990201621, 9.18075260120879, 9.13651001887094, 9.09234307598404, 9.04825269180332, 9.0042397815232, 8.96030525376274, 8.91645000786404, 8.87267493099424, 8.8289808950396, 8.78536875328062, 8.74183933683067, 8.69839345081615, 8.65503187027711, 8.61175533575459, 8.56856454852898, 8.52546016546591, 8.48244279341313, 8.43951298309221, 8.39667122240631, 8.35391792908569, 8.31125344257359, 8.26867801504638, 8.22619180145052, 8.18379484842406, 8.14148708196249, 8.09926829367804, 8.05713812549137, 8.01509605259222, 7.97314136450051, 7.93127314406215, 7.88949024421893, 7.84779126240348, 7.8061745124266, 7.7646379937456, 7.72317935802947, 7.68179587296812, 7.64048438330365, 7.59924126909409, 7.55806240124589, 7.51694309436604, 7.47587805698376, 7.4348613391631, 7.39388627746716, 7.35294543712698, 7.31203055110922, 7.27113245554973, 7.23024102072137, 7.18934507632427, 7.14843232941731, 7.10748927277792, 7.06650108328555, 7.0254514913046, 6.98432265556781, 6.94309498601845, 6.90174694757117, 6.86025482165158, 6.81859241756945, 6.77673073566965, 6.73463754091527, 6.6922768727898, 6.64960844666737, 6.60658693578496, 6.56316111114983, 6.51927280454337, 6.47485565402908, 6.4298335753112, 6.38411888189302, 6.33760994856354, 6.29018827347556, 6.24171473691697, 6.19202476558075, 6.1409219673242, 6.08816957309651, 6.0334786654947, 5.97649160131111, 5.91675806354951, 5.85369941530768, 5.78655363305194, 5.7142861171291, 5.63543603228236, 5.54782844912054, 5.44796678240509, 5.32949618331455, 5.1779036068329, 4.9322404466402, 4.61575056360921, 4.65794459831218, 4.68581554950078, 4.70167757295937, 4.71852141284815, 4.74155551062613, 4.76334906217805, 4.78166236903416, 4.79452855556043, 4.80001265069886, 4.79676020476811, 4.78502740813599, 4.76764910487257; 9.52360240965362, 9.47769843542883, 9.43186175495492, 9.38609323987884, 9.34039376317769, 9.29476419725495, 9.24920541187706, 9.20371827194226, 9.15830363507413, 9.11296234903031, 9.06769524891492, 9.02250315418351, 8.97738686542358, 8.93234716088999, 8.88738479277489, 8.84250048318102, 8.79769491976513, 8.75296875101128, 8.70832258108238, 8.66375696419804, 8.61927239846716, 8.57486931910301, 8.53054809093204, ...(+40714 chars)] kJ/(K*kg)  T_vap=[280.119570224693, 281.817374107986, 283.538600806196, 285.283770454129, 287.053419505052, 288.848101348403, 290.668386956629, 292.514865562118, 294.388145365577, 296.288854277168, 298.217640691671, 300.175174299661, 302.162146936045, 304.179273467418, 306.227292720712, 308.306968454521, 310.419090375271, 312.56447520062, 314.743967771488, 316.958442216232, 319.208803168108, 321.495987039359, 323.820963354129, 326.184736142855, 328.588345401182, 331.03286861587, 333.519422360829, 336.049163966471, 338.623293265115, 341.243054415991, 343.909737812947, 346.624682078325, 349.389276146405, 352.204961439991, 355.073234143788, 357.995647578143, 360.973814677087, 364.009410574379, 367.104175301498, 370.259916601442, 373.478512862336, 376.761916174597, 380.112155515582, 383.531340065176, 387.021662655815, 390.585403359598, 394.224933214993, 397.942718094376, 401.741322712673, 405.623414775823, 409.591769265657, 413.649272855207, 417.798928445221, 422.043859808325, 426.387316322197, 430.832677766469, 435.383459150095, 440.043315525875, 444.816046736328, 449.705602019631, 454.716084384802, 459.851754640606, 465.117034931359, 470.516511592278, 476.054937084766, 481.737230703455, 487.568477656811, 493.553926003915, 499.698980772256, 506.009194370097, 512.490252121224, 519.147951355182, 525.988171934846, 533.016835328216, 540.239848239874, 547.663025262204, 555.291982729155, 563.13199248708, 571.187778762452, 579.463231984088, 587.960996709728, 596.681859170256, 605.623800233703, 614.780487495712, 624.138943840341, 633.675949835929, 643.335370256395, 653.176316245141, 663.669120579666, 674.581895018015, 685.634225017016, 697.095645012442, 709.33376966421, 722.043885341972, 735.01024973374, 747.930800167236, 760.410061546282, 772.034275421014, 782.553470870924, 792.122247735498; 327.733744381795, 329.328564401229, 330.94450069677, 332.58199563221, 334.241503992079, 335.923493299301, 337.628444146888, 339.356850545858, 341.109220292044, 342.886075354511, 344.687952288365, 346.515402675313, 348.368993594682, 350.249308127411, 352.156945896287, 354.092523644071, 356.05667585147, 358.050055396286, 360.073334253411, 362.127204236296, 364.212377777219, 366.32958874474, 368.479593294229, 370.66317074685, 372.88112449154, 375.134282903131, 377.423500269823, 379.749657723097, 382.113664163239, 384.516457175725, 386.959003935628, 389.442302101198, 391.967380702838, 394.535301040759, 397.147157613522, 399.804079110581, 402.507229515038, 405.25780937814, 408.057057343445, 410.906252016711, 413.806714295746, 416.75981029161, 419.766954987692, 422.829616793638, 425.949323155628, 429.127667379594, 432.366316808589, 435.667022465672, 439.031630228684, 442.462093541092, 445.960487583167, 449.529024730918, 453.170070955048, 456.886163154306, 460.680025907675, 464.554588304517, 468.512999132413, 472.558639972257, 476.695135345028, 480.92635851415, 485.256433374436, 489.68973015775, 494.230854803967, 498.884633038041, 503.656086401072, 508.550402017206, 513.572895205184, 518.728964757739, 524.024040264263, 529.463520510755, 535.05270173828, 540.796694103574, 546.70032321406, 552.768010212996, 559.003618733281, 565.410251615595, 571.989975794075, 578.743448726219, 585.66940935902, 592.763973379138, 600.01962322215, 607.42367253603, 614.95569967493, 622.582604997472, 630.247058108915, 637.831386075871, 644.95486208936, 653.907399970642, 665.742753937643, 678.050904902505, 690.480249792388, 703.256357842723, 716.745136589454, 730.647760810727, 744.745107398519, 758.736520846055, 772.234133009228, 784.835133089508, 796.298805903605, 806.779630534537; 375.071153960372, 376.572096107005, 378.09243323305, 379.632549528416, 381.192838781726, 382.773704547385, 384.375560317838, 385.998829702581, 387.64394661579, 389.311355474567, 391.00151140965, 392.714880491056, 394.451939970335, 396.213178540908, 397.999096618569, 399.810206642603, 401.647033398173, 403.510114359911, 405.400000054933, 407.31725444434, 409.262455318881, 411.236194705408, 413.239079278115, ...(+40739 chars)] K  nu_vap=[1181.7506820838, 1064.70727047747, 959.379071262689, 864.582180888748, 779.253385028805, 702.437755591613, 633.277532125753, 571.002153627892, 514.91932084744, 464.406981767999, 418.906144203296, 377.914429515304, 340.98029046474, 307.697824260462, 277.702119082886, 250.665078801251, 226.291676376064, 204.316591600875, 184.50119345683, 166.630831492364, 150.512404338974, 135.972176791541, 122.853819847245, 111.016650754853, 100.334052505683, 90.6920543279329, 81.9880566551476, 74.1296857490858, 67.0337646884604, 60.625388807574, 54.8370948979486, 49.6081145878511, 44.8837033017932, 40.6145370869456, 36.7561703864877, 33.2685485508139, 30.1155695149283, 27.2646896417428, 24.6865692433917, 22.3547537521527, 20.2453869246526, 18.3369528326127, 16.6100437249742, 15.0471511436442, 13.6324779420149, 12.3517690948497, 11.1921594030994, 10.142036390094, 9.19091685875611, 8.32933573497455, 7.54874596188392, 6.84142833518883, 6.20041028227126, 5.61939268894499, 5.09268396854783, 4.61514064961552, 4.18211383161123, 3.78940092391797, 3.43320214228913, 3.11008128987423, 2.81693039739238, 2.55093783956501, 2.30955958303697, 2.09049325514859, 1.89165475347617, 1.71115714339149, 1.54729161534465, 1.39851029547319, 1.26341072278225, 1.1407218236957, 1.02929123018807, .928073800661277, .83612121293809, .75257250622596, .676645453859501, .607628650423765, .544874192547012, .4877908154527, .43583730394362, .388515897922535, .345365184992008, .305951404083241, .269855500495175, .23664823361107, .205826260329913, .176579581337147, .14630245920675, .125467572432497, .125734621578621, .12644897390339, .126865576214116, .127361970298116, .128075646075567, .128702663574326, .129152436711277, .129359560914246, .129285446195106, .128941286656531, .128412654616677, .127855447803605; 1617.30601851652, 1454.93708149042, 1308.99399578077, 1177.80383345005, 1059.86505715481, 953.829868914358, 858.488385482276, 772.754450448677, 695.652913023187, 626.308221190342, 563.934192813096, 507.824842483148, 457.346154646159, 411.928704931413, 371.061041826585, 334.283749975856, 301.18412456877, 271.391393618352, 244.572431491763, 220.427912941364, 198.688862147758, 179.113556008837, 161.484745133559, 145.607159787, 131.305271425881, 118.421283502739, 106.813327941018, 96.3538461234914, 86.9281354229022, 78.4330442638572, 70.7758004608829, 63.8729591517612, 57.6494580559477, 52.037769052484, 46.9771362053356, 42.4128913802212, 38.2958395080054, 34.5817063665317, 31.2306424850115, 28.206777431837, 25.4778193355846, 23.01469501714, 20.7912265847154, 18.7838407685738, 16.9713076537482, 15.3345058113627, 13.8562111365538, 12.5209069769361, 11.3146133834522, 10.224733538119, 9.23991561322702, 8.34992849674036, 7.54555002017048, 6.81846617285815, 6.16118083416494, 5.56693410992716, 5.02962905506951, 4.54376568633162, 4.10438158399562, 3.70699853455794, 3.34757434759919, 3.02245968678382, 2.72835916713259, 2.46229635720672, 2.22158233473892, 2.00378739340552, 1.80671559587713, 1.62838187482152, 1.46699141335821, 1.32092106221591, 1.18870257564118, 1.06900746899799, .96063331367374, .862491288539338, .773594807493042, .693049046415235, .620041197023111, .553831260790013, .493743132742124, .439155568384721, .389492280189213, .344209587319944, .302777821740958, .264645729010402, .229150343813528, .195188783326182, .158748822997459, .131735584113327, .13231727848491, .132783228464214, .13278945698941, .132914019134807, .133337443852661, .133670673459254, .133804349710562, .133666142230286, .133216365489149, .132471574091176, .131530896028188, .130571213283232; 2147.51662378051, 1929.05308474225, 1732.95041421399, 1556.90748842306, 1398.86110088829, 1256.96126203826, 1129.5490727679, 1015.13690278695, 912.390632849301, 820.11374521479, 737.233069300409, 662.786009709324, 595.909101925293, 535.82775716155, 481.847072355187, 433.343594270209, 389.757938289717, 350.588172873003, 315.38388995666, 283.740889912129, 255.296417123698, 229.724888930016, 206.734066645332, ...(+40723 chars)] mm^2/s  k_vap=[.0172121806918844, .0173239896506616, .0174380026922971, .0175542852788582, .0176729059668326, .0177939366312882, .017917452709536, .0180435334659969, .0181722622801357, .0183037269594715, .0184380200798319, .0185752393552424, .0187154880399796, .0188588753655271, .0190055170154588, .0191555356414236, .0193090614237156, .0194662326801918, .0196271965275172, .0197921095991826, .019961138824903, .0201344622765296, .0203122700859208, .0204947654406838, .0206821656641993, .0208747033868162, .0210726278157276, .0212762061116746, .0214857248812934, .0217014917947741, .0219238373393471, .0221531167201427, .0223897119211026, .0226340339399283, .0228865252125558, .0231476561584934, .023417950894082, .0236979579130179, .023988273991347, .0242895429635371, .0246024597220271, .0249277745813578, .0252662980476687, .0256189060407188, .0259865456233571, .0263702413027666, .026771101979405, .0271903286338259, .0276292228593632, .0280891963709871, .0285717816488581, .0290786439111082, .0296115946566485, .0301726070787337, .0307638337282867, .0313876269089436, .0320465624222649, .0327434674638099, .0334814537159306, .0342639570154336, .0350947854281118, .0359781781871146, .036918878820204, .0379222270080118, .0389942754392702, .0401419403979816, .041373198397564, .0426973464396154, .0441253513293925, .0456703253989442, .0473481843996195, .0491785723141815, .0511861844710541, .0534026972260988, .0558696427991561, .0586427955292582, .06179904676714, .065447514794826, .0697481370702856, .0749440680896103, .0814208963897291, .0898213950322921, .101285449253741, .118009758569914, .144813615914794, .195387606958831, .356836775307517, .46583411910122, .359796128727985, .324876439027368, .31064671079789, .305269431763675, .303181776191216, .304314229552229, .308328652118479, .315119418755774, .32470127809822, .337039993160857, .351837536465925, .36837563811304; .0205738712416131, .0206941697420259, .0208165864984598, .0209411791394681, .0210680077930817, .0211971352448655, .0213286271096266, .0214625520181484, .0215989818204838, .0217379918074666, .0218796609522415, .0220240721738122, .0221713126247106, .0223214740050557, .0224746529055166, .0226309511817721, .022790476363306, .0229533420995663, .0231196686466443, .0232895833979876, .0234632214627014, .023640726295406, .0238222503817845, .0240079559843014, .0241980159529462, .0243926146062179, .0245919486881091, .0247962284074354, .0250056785665364, .0252205397873124, .0254410698435914, .0256675451101592, .0259002621403693, .0261395393861876, .026385719076848, .0266391692750522, .0269002861328967, .0271694963735256, .0274472600288376, .0277340734685533, .0280304704039571, .0283370343891083, .0286543906666046, .0289832185833645, .0293242549802763, .0296783000562598, .0300462239554009, .0304289741713051, .0308275838728573, .0312431812670356, .0316770001281731, .0321303916404087, .0326048377097454, .0331019660303565, .0336235669458529, .0341716126853446, .0347482791706924, .0353559709944755, .0359973502673926, .036675370151315, .0373933146179559, .0381548457908977, .0389640613807202, .0398255655309171, .0407445571648308, .0417269421174738, .0427794773878485, .0439099593758531, .0451274729792489, .0464427259470321, .0478685043386672, .0494203026965547, .0511172106800478, .0529831837324597, .0550489022684621, .0573545570619634, .0599541368772989, .0629222373803286, .0663652714224833, .0704407256166943, .0753919617460742, .0816151622442414, .0897988325032829, .101248239843368, .118778483398841, .150065162836688, .236616384202989, .394217174599135, .313920177737169, .287138615166654, .277825854774133, .274989919322927, .274872749304205, .277835525113959, .283545705873854, .291865904898272, .302784031168293, .3162496497754, .331974376910159, .349288586075868; .0243189758743705, .0244442036796683, .0245714610788146, .0247007992854865, .0248322715298354, .0249659331743534, .0251018418396998, .0252400575415492, .0253806428396502, .0255236630003846, .0256691861742272, .0258172835896719, .0259680297652603, ...(+42254 chars)] W/(K*m)  Pr_vap=[1.00530779386979, 1.00527931100127, 1.00527774677782, 1.00530215602599, 1.00535168776081, 1.00542560542535, 1.00552330745334, 1.00564434786696, 1.00578845660751, 1.00595555929195, 1.00614579609427, 1.00635953946623, 1.00659741044364, 1.00686029333183, 1.00714934861932, 1.00746602405339, 1.00781206390221, 1.00818951654268, 1.00860074064224, 1.0090484103457, 1.00953552003959, 1.01006538942343, 1.01064166979877, 1.01126835264281, 1.01194978169218, 1.01269066989353, 1.01349612267036, 1.01437166899855, 1.01532330175571, 1.01635752869034, 1.01748143512898, 1.01870275917818, 1.02002997966656, 1.02147241639336, 1.02304034139593, 1.02474536833867, 1.02659956257514, 1.02861701030618, 1.03081302232638, 1.03320445933677, 1.03580981632782, 1.03864927502842, 1.04174471408665, 1.04511966671828, 1.04879921644953, 1.05280982348908, 1.05717907737094, 1.0619353759444, 1.06710753661823, 1.07272435295754, 1.07881411813593, 1.08540414607038, 1.0925203308794, 1.1001867950328, 1.10842568551885, 1.11725718479211, 1.12669980844603, 1.13677106384393, 1.14748854294511, 1.15887151824741, 1.17094310363291, 1.18373303311534, 1.1972811019733, 1.21164130916731, 1.22688674062855, 1.24311524467346, 1.26045598214144, 1.27907700142644, 1.2991941146049, 1.32108154540288, 1.34508505886212, 1.3716385337835, 1.40128527075306, 1.43470601968056, 1.4727571946079, 1.51652542510248, 1.56740896595161, 1.62724406333563, 1.6985098353461, 1.78468131606412, 1.89089274941351, 2.02533394435917, 2.20263229877464, 2.45356624441721, 2.86005365869031, 3.73995770157405, 8.49228931516112, 12.7774049886644, 5.40646761311355, 3.55157467027475, 2.68691879613355, 2.19689670808065, 1.87632480536004, 1.64357285741673, 1.46520221075526, 1.32329612246206, 1.20700834546265, 1.10975650037544, 1.02760086674803, .958115213107679; .975820082604012, .975599638448165, .975389470379557, .975190034110188, .975001811842088, .97482531318137, .974661076079447, .974509667809326, .974371685986989, .974247759650502, .974138550412616, .974044753706008, .973967100144761, .97390635703056, .973863330037527, .973838865116564, .973833850667507, .973849220036163, .973885954403756, .973945086147312, .974027702763632, .974134951463962, .974268044564328, .974428265815965, .974616977842587, .974835630876605, .975085773014667, .975369062244596, .975687280531639, .976042350290993, .976436353617495, .976871554690826, .977350425827925, .977875677709372, .978450294369401, .979077573603742, .979761173518939, .980505166019988, .981314098109456, .982193061950223, .983147857414659, .984184774545559, .9853111313436, .986535116113012, .987865983675718, .989314202836935, .990891621720082, .99261165267127, .994489478571555, .996542282567367, .998789503455409, 1.00125311926425, 1.00395796173736, 1.00693206699386, 1.01020706267757, 1.01381860292568, 1.01780685466508, 1.02221704712121, 1.02710009851118, 1.03251333691701, 1.03852134609914, 1.04519696506123, 1.05262249450267, 1.0608911722363, 1.0701090063837, 1.08039708170717, 1.09189449328154, 1.10476211091815, 1.11918744596025, 1.13539098983545, 1.15363453829781, 1.17423223286891, 1.19756538411029, 1.22410266298553, 1.25442808575756, 1.28928061209149, 1.32961159055257, 1.37667069631947, 1.43213960248075, 1.4983507314809, 1.57867033266605, 1.67823392009625, 1.8055468838585, 1.97661596530431, 2.22845520752916, 2.68317181287304, 4.32508157005078, 9.01847711310476, 4.66115985009522, 3.30632907866698, 2.62976444882911, 2.1982578905111, 1.89401975289029, 1.6675745907044, 1.49126295620293, 1.34893872744833, 1.23085564998631, 1.13104353132813, 1.04594295587745, .973462585945187; .965390719678975, .965187004652924, .964985067143916, .964785092635174, .964587280949934, .964391847165687, .96419902258883, .96400905579639, .963822213752743, .96363878301059, .963459071007211, .963283407468869, .963112145938666, .962945665445906, .962784372338036, .962628702300189, .962479122591557, .962336134532904, .962200276285541, .962072125968678, .9619523051701, .961841482914291, .961740380162418, ...(+40744 chars)]  u_sat_vap=[2384.48887142334; 2386.8190727186; 2389.17956798209; 2391.57090439466; 2393.99363630932; 2396.44832463482; 2398.93553613589; 2401.45584264345; 2404.00982016729; 2406.59804790336; 2409.22110712587; 2411.87957995478; 2414.5740479859; 2417.30509076955; 2420.07328412268; 2422.87919825479; 2425.72339568653; 2428.60642893589; 2431.52883794202; 2434.49114719473; 2437.49386252932; 2440.53746754394; 2443.62241958864; 2446.74914526951; 2449.91803540424; 2453.12943935745; 2456.38365867683; 2459.68093994327; 2463.02146673929; 2466.40535063317; 2469.83262106808; 2473.30321403865; 2476.81695943156; 2480.37356690123; 2483.97261014837; 2487.6135094662; 2491.29551241775; 2495.01767250802; 2498.77882571352; 2502.57756473221; 2506.4122108135; 2510.28078302177; 2514.18096477359; 2518.11006746621; 2522.06499097839; 2526.04218077002; 2530.0375812296; 2534.04658481179; 2538.0639763666; 2542.08387188043; 2546.09965062185; 2550.10387940661; 2554.08822736159; 2558.0433691714; 2561.95887432961; 2565.82307938264; 2569.62293953897; 2573.34385530705; 2576.96946899843; 2580.48142495507; 2583.85908617711; 2587.07919855877; 2590.11549206752; 2592.93820574884; 2595.51352014923; 2597.80287623098; 2599.76215352509; 2601.34067132824; 2602.47996418797; 2603.11226548206; 2603.15860857737; 2602.52641976574; 2601.1064230059; 2598.76859062443; 2595.35673813697; 2590.68114690764; 2584.50825239438; 2576.54584814744; 2566.42119590362; 2553.64740422076; 2537.56929184321; 2517.27071175594; 2491.40220665335; 2457.82041689229; 2412.68530445105; 2347.38049805772; 2226.48555738068; 2056.34806264226; 2088.50059191893; 2112.4350204755; 2129.37026909632; 2147.13438479139; 2169.16824543376; 2190.91474512801; 2210.90554944606; 2227.7371454335; 2239.91027703293; 2246.22462783334; 2246.56933058969; 2242.74587564859] kJ/kg
      settings: InternalSimscapePortConfiguration="{\"Bottom\":[],\"Left\":[],\"Right\":[{\"id\":\"A\",\"label\":\"\",\"type\":\"foundation.two_phase_fluid.two_phase_fluid\"}],\"Top\":[]}"
  Two-Winding Transformer (Three-Phase) : ee_lib/Passive/Transformers/Two-Winding Transformer (Three-Phase)  SRated=15E6 A*V  FRated=60 Hz  Winding1Connection=ee.enum.windingconnection.delta1  VRated1=24E3 V  Winding2Connection=ee.enum.windingconnection.Yg  VRated2=138e3 V  CoreType=ee.enum.coretype.threelimb  pu_Rw1=0.01  pu_Rw2=0.01  leakage_reactance_option=ee.enum.transformer_leakage.exclude  pu_Xl1=0.05  pu_Xl2=0.05  magnetizing_resistance_option=ee.enum.transformer_magnetizingResistance.exclude  pu_Rm=500  magnetizing_reactance_option=ee.enum.transformer_magnetizingReactance.exclude  saturation_option=ee.enum.transformer_saturation.exclude  pu_Xm=500  current_data=[0, .002, 1, 2]  magnetic_flux_data=[0, 1.2, 1.5, 1.51]  pu_X0=0.5  i1_specify=off  i1_priority=None  i1=[0, 0, 0] A  i1_nominal_specify=off  i1_nominal_unit=A  i1_nominal_value=1  i2_specify=off  i2_priority=None  i2=[0, 0, 0] A  i2_nominal_specify=off  i2_nominal_unit=A  i2_nominal_value=1  phi_specify=off  phi_priority=None  phi=[0, 0, 0]  phi_nominal_specify=off  phi_nominal_unit=1  phi_nominal_value=1  power_dissipated_specify=off  power_dissipated_priority=None  power_dissipated=0 W  power_dissipated_nominal_specify=off  power_dissipated_nominal_unit=W  power_dissipated_nominal_value=1
      settings: InternalSimscapePortConfiguration="{\"Bottom\":[],\"Left\":[{\"id\":\"N1\",\"label\":\"~1\",\"type\":\"foundation.electrical.three_phase\"}],\"Right\":[{\"id\":\"N2\",\"label\":\"~2\",\"type\":\"foundation.electrical.three_phase\"}],\"Top\":[]}"
  Vapor Quality Sensor (2P){1..4} (4 alike) : fl_lib/Two-Phase Fluid/Sensors/Vapor Quality Sensor (2P)  vapor_fraction_spec=foundation.enum.vapor_fraction_spec.quality
      settings: InternalSimscapePortConfiguration="{\"Bottom\":[],\"Left\":[{\"id\":\"A\",\"label\":\"A\",\"type\":\"foundation.two_phase_fluid.two_phase_fluid\"}],\"Right\":[{\"id\":\"X\",\"label\":\"X\",\"type\":\"output\"}],\"Top\":[]}"
  Variable-Displacement Pump (2P) : SimscapeFluids_lib/Two-Phase Fluid/Fluid Machines/Variable-Displacement Pump (2P)  leakage_friction_spec=fluids.two_phase_fluid.fluid_machines.enum.PumpMotorLossSpec.Analytical  displacement_nominal=8.33e-6 * 2 m^3/rev  omega_nominal=525 rad/s  p_nominal=5 MPa  mu_nominal=0.3 cP  vol_eff_nominal=0.92  mech_eff_nominal=0.88  no_load_torque=0 N*m  p_diff_eff_TLU=[.1, 1, 2] MPa  omega_eff_TLU=[25, 50, 100, 200, 300, 400] rad/s  displacement_eff_TLU=[-30, -19, 19, 30] cm^3/rev  vol_eff_TLU=repmat([.816, .908, .954, .977, .981, .984; .325, .663, .831, .916, .925, .946; .137, .568, .78, .892, .893, .91], 1, 1, 4)  mech_eff_TLU=repmat([.996, .996, .996, .996, .996, .996; .988, .989, .989, .989, .989, .99; .981, .981, .982, .982, .983, .984], 1, 1, 4)  p_diff_loss_TLU=[.1, 1, 2] MPa  omega_loss_TLU=[25, 50, 100, 200, 300, 400] rad/s  displacement_loss_TLU=[-30, -19, 19, 30] cm^3/rev  vol_loss_TLU=repmat(1e-3 * [.023, .023, .023, .023, .0285, .032; .0844, .0842, .0845, .084, .1125, .108; .1079, .108, .11, .108, .1605, .18], 1, 1, 4) m^3/s  mech_loss_TLU=repmat([.002, .002, .002, .002, .002, .002; .0607, .0556, .0556, .0556, .0556, .0505; .1937, .1937, .1833, .1833, .1729, .1626], 1, 1, 4) N*m  vol_eff_min=1e-3  vol_eff_max=1  mech_eff_min=1e-3  mech_eff_max=1  pressure_threshold=1e-3 MPa  omega_threshold=10 rad/s  displacement_threshold=0.1 cm^3/rev  area=2.03E-3 m^2  liquid_check=simscape.enum.assert.action.none  octant_check=simscape.enum.assert.action.none  pump_mode_check=simscape.enum.assert.action.none
      settings: InternalSimscapePortConfiguration="{\"Bottom\":[{\"id\":\"A\",\"label\":\"A\",\"type\":\"foundation.two_phase_fluid.two_phase_fluid\"}],\"Left\":[{\"id\":\"D\",\"label\":\"D\",\"type\":\"input\"}],\"Right\":[{\"id\":\"R\",\"label\":\"R\",\"type\":\"foundation.mechanical.rotational.rotational\"},{\"id\":\"C\",\"label\":\"C\",\"type\":\"foundation.mechanical.rotational.rotational\"}],\"Top\":[{\"id\":\"B\",\"label\":\"B\",\"type\":\"foundation.two_phase_fluid.two_phase_fluid\"}]}"
  wires:
  PS-Simulink Converter17/1 -> Display17/1
  Add2/1 -> Heat Removed/1
  Subtract2/1 -> Qsg/1
  Product3/1 -> Add1/1
  PS-Simulink Converter9/1 -> Display8/1
  PS-Simulink Converter15/1 -> Display14/1
  PS-Simulink Converter49/1 -> Display50/1
  Subtract1/1 -> Product1/1
  [Phi_sg_in] -> Subtract2/2
  PS-Simulink Converter14/1 -> Display13/1
  PS-Simulink Converter27/1 -> Display27/1
  Constant2/1 -> Switch1/1
  PS-Simulink Converter12/1 -> Display12/1
  [L] -> Subtract1/2, Product2/2
  [Mdot_prim] -> Subsystem/2(In2)
  PS-Simulink Converter8/1 -> Display6/1
  PS-Simulink Converter18/1 -> Display18/1
  PS-Simulink Converter53/1 -> Display54/1
  Product2/1 -> Product4/1
  [P_err] -> Preheating/1(In1)
  PS-Simulink Converter38/1 -> Display39/1
  PS-Simulink Converter1/1 -> [T_react], Display1/1
  Switch/1 -> [LoopReady], Simulink-PS Converter2/1, Display55/1
  PS-Simulink Converter26/1 -> Display26/1
  PS-Simulink Converter25/1 -> Display25/1
  PS-Simulink Converter52/1 -> Display53/1
  Product/1 -> Abs/1
  PS-Simulink Converter59/1 -> [Phi_sg_out], Display64/1
  PS-Simulink Converter40/1 -> Display41/1
  Gain1/1 -> Display59/1, [Pshaft_HP]
  PS-Simulink Converter56/1 -> Display61/1, Product4/2
  PS-Simulink Converter21/1 -> Display21/1
  Discrete Transfer Fcn3/1 -> Display86/1, Simulink-PS Converter3/1
  Subtract3/1 -> Add2/1, Qcond/1
  [P_drum] -> Startup Controller/3(Drum Pressure)
  Saturation1/1 -> Display58/1, Simulink-PS Converter1/1
  Product5/1 -> Abs1/1
  Subtract/1 -> Discrete PID Controller/1
  Gain2/1 -> [Pshaft_IP], Display85/1
  PS-Simulink Converter50/1 -> Display51/1
  [LoopReady] -> Switch1/2
  PS-Simulink Converter3/1 -> [T_sg], Display3/1
  PS-Simulink Converter68/1 -> Display74/1
  Switch1/1 -> Discrete Transfer Fcn1/1
  PS-Simulink Converter66/1 -> Display71/1, Product5/2
  PS-Simulink Converter74/1 -> Display80/1
  PS-Simulink Converter78/1 -> Product5/1, Display84/1
  Abs1/1 -> Gain2/1
  Constant1/1 -> Add/1
  PS-Simulink Converter55/1 -> Display57/1
  PS-Simulink Converter72/1 -> Display78/1
  Clock/1 -> Switch/2
  PS-Simulink Converter23/1 -> Display23/1
  PS-Simulink Converter/1 -> [P_err], Display/1
  PS-Simulink Converter31/1 -> Display32/1
  PS-Simulink Converter58/1 -> Display63/1
  [T_sg] -> Preheating/3(In2)
  Add1/1 -> Display62/1
  PS-Simulink Converter4/1 -> [mdot_scndry], Display5/1
  PS-Simulink Converter16/1 -> Display15/1
  Saturation/1 -> Discrete Transfer Fcn/1
  PS-Simulink Converter22/1 -> [P_down], Display22/1
  PS-Simulink Converter41/1 -> Display42/1
  PS-Simulink Converter19/1 -> Display19/1
  Band-Limited White Noise/1 -> Gain/1
  Add/1 -> Switch1/3
  Discrete Transfer Fcn1/1 -> Saturation1/1
  [Phi_cond_out] -> Subtract3/2
  [mdot_scndry] -> Subtract/2
  PS-Simulink Converter6/1 -> Display7/1
  PS-Simulink Converter47/1 -> Product/1, Display48/1
  PS-Simulink Converter10/1 -> [Wdot_in], Display30/1
  PS-Simulink Converter51/1 -> Display52/1
  [Gen_Real_Power] -> Startup Controller/2(Generator Real Power)
  PS-Simulink Converter30/1 -> Display31/1
  [Press_primary] -> Subsystem/1(In1)
  Discrete Transfer Fcn/1 -> Display9/1, Simulink-PS Converter/1
  PS-Simulink Converter54/1 -> Display56/1
  PS-Simulink Converter11/1 -> Display10/1
  PS-Simulink Converter57/1 -> Display60/1, Product3/1
  PS-Simulink Converter46/1 -> Display47/1
  PS-Simulink Converter5/1 -> Display16/1, [L]
  Constant5/1 -> Switch/3
  [P_demand] -> Startup Controller/1(Grid Demand)
  PS-Simulink Converter60/1 -> [Phi_sg_in], Display65/1
  PS-Simulink Converter2/1 -> Display2/1
  Gain/1 -> Discrete Transfer Fcn2/1
  PS-Simulink Converter71/1 -> Display77/1
  PS-Simulink Converter64/1 -> [Mdot_prim], Display70/1
  Abs/1 -> Gain1/1
  PS-Simulink Converter62/1 -> Subtract4/1, Display67/1
  [Phi_sg_out] -> Subtract2/1
  PS-Simulink Converter37/1 -> Display38/1
  PS-Simulink Converter70/1 -> Display76/1
  Add3/1 -> Display87/1, Add2/2
  PS-Simulink Converter65/1 -> Display72/1
  PS-Simulink Converter73/1 -> Display79/1
  Discrete PID Controller/1 -> Saturation/1
  PS-Simulink Converter29/1 -> [Phi_cond_in], Display29/1
  [Pshaft_HP] -> Add3/1
  PS-Simulink Converter67/1 -> Display73/1
  PS-Simulink Converter45/1 -> Display46/1
  PS-Simulink Converter80/1 -> Display89/1
  Constant4/1 -> Switch/1
  PS-Simulink Converter69/1 -> Display75/1
  [Phi_cond_in] -> Subtract3/1
  [Pshaft_LP] -> Add3/2
  Constant6/1 -> Subtract1/1
  PS-Simulink Converter24/1 -> Display24/1
  PS-Simulink Converter61/1 -> [Phi_cond_out], Display66/1
  PS-Simulink Converter44/1 -> Display45/1
  Constant/1 -> Subtract/1
  PS-Simulink Converter7/1 -> Display4/1
  Startup Controller/1(Vt) -> [Vt]
  PS-Simulink Converter34/1 -> Display35/1
  Constant3/1 -> Product2/1, Product1/2
  PS-Simulink Converter28/1 -> Display28/1
  Subtract4/1 -> Display69/1
  PS-Simulink Converter63/1 -> Subtract4/2, Display68/1
  PS-Simulink Converter43/1 -> Display44/1
  Product1/1 -> Product3/2
  PS-Simulink Converter42/1 -> Display43/1
  PS-Simulink Converter48/1 -> [Gen_Real_Power], Display49/1
  PS-Simulink Converter75/1 -> Display81/1
  Product4/1 -> Add1/2
  PS-Simulink Converter77/1 -> Display83/1
  PS-Simulink Converter32/1 -> Display33/1
  PS-Simulink Converter13/1 -> Display11/1, Product/2
  PS-Simulink Converter39/1 -> Display40/1, [Press_primary]
  PS-Simulink Converter35/1 -> Display36/1
  PS-Simulink Converter79/1 -> Display88/1
  Constant7/1 -> Discrete Transfer Fcn3/1
  PS-Simulink Converter36/1 -> Display37/1
  PS-Simulink Converter76/1 -> Display82/1
  PS-Simulink Converter33/1 -> Display34/1
  PS-Simulink Converter20/1 -> [P_drum], Display20/1
  [T_react] -> Subsystem1/1(In1)
  PS-Simulink Converter81/1 -> Display90/1
  PS-Simulink Converter95/1 -> Product6/1, Display104/1
  PS-Simulink Converter82/1 -> Display92/1
  PS-Simulink Converter87/1 -> Display96/1
  PS-Simulink Converter89/1 -> Display98/1
  PS-Simulink Converter85/1 -> Display94/1
  Abs2/1 -> Gain3/1
  PS-Simulink Converter91/1 -> Display100/1
  Gain3/1 -> [Pshaft_LP], Display105/1
  PS-Simulink Converter94/1 -> Display103/1
  PS-Simulink Converter90/1 -> Display99/1
  PS-Simulink Converter92/1 -> Display101/1
  PS-Simulink Converter84/1 -> Display93/1
  PS-Simulink Converter83/1 -> Display91/1, Product6/2
  Product6/1 -> Abs2/1
  PS-Simulink Converter93/1 -> Display102/1
  PS-Simulink Converter86/1 -> Display95/1
  PS-Simulink Converter88/1 -> Display97/1
  Constant8/1 -> Discrete Transfer Fcn4/1
  Discrete Transfer Fcn4/1 -> Display106/1, Simulink-PS Converter4/1
  Discrete Transfer Fcn5/1 -> Simulink-PS Converter5/1, Display107/1
  Constant9/1 -> Discrete Transfer Fcn5/1
  [Pshaft_IP] -> Add3/3
  [Press_primary] -> Subsystem1/2(In2)
  Constant10/1 -> Simulink-PS Converter6/1
  PS-Simulink Converter96/1 -> Display108/1
  PS-Simulink Converter97/1 -> Display109/1
  PS-Simulink Converter98/1 -> Display110/1
  PS-Simulink Converter99/1 -> Display111/1
  PS-Simulink Converter100/1 -> Display112/1
  PS-Simulink Converter102/1 -> Display114/1
  PS-Simulink Converter101/1 -> Display113/1
  connections:
  Steam Generator/LConn2 -- Centrifugal Pump (TL)/LConn1 -- Pressure & Temperature Sensor (TL)1/LConn1 -- Solver Configuration/RConn1 -- Thermal Liquid Properties (TL)/RConn1
  Thermodynamic Properties Sensor (2P)3/LConn1 -- Vapor Quality Sensor (2P)4/LConn1 -- Simscape Component2/LConn2 -- Mass & Energy Flow Rate Sensor (2P)4/RConn1 -- Mass & Energy Flow Rate Sensor (2P)2/LConn1 -- Pressure & Internal Energy Sensor (2P)1/LConn1
  Pressure & Temperature Sensor (TL)2/LConn1 -- Mass & Energy Flow Rate Sensor (TL)3/LConn1 -- Pipe (TL)2/RConn1 -- Steam Generator/LConn1
  Thermodynamic Properties Sensor (2P)/LConn1 -- Mass & Energy Flow Rate Sensor (2P)8/RConn1 -- Steam Generator/RConn1 -- Check Valve (2P)2/RConn1
  Simscape Component1/RConn2 -- Simscape Component2/RConn2 -- Synchronous Machine Round Rotor/LConn4 -- Mechanical Rotational Reference2/LConn1 -- Simscape Component/RConn2
  Mass & Energy Flow Rate Sensor (2P)/LConn1 -- Variable-Displacement Pump (2P)/LConn2 -- Pressure & Internal Energy Sensor (2P)/LConn1
  Pressure & Temperature Sensor (TL)/LConn1 -- Pipe (TL)2/LConn1 -- Pipe (TL)/RConn1
  Two-Phase Fluid Properties (2P)/RConn1 -- Pressure & Internal Energy Sensor (2P)4/LConn1 -- Vapor Quality Sensor (2P)1/LConn1 -- Thermodynamic Properties Sensor (2P)1/LConn1 -- Steam Drum/LConn1 -- Mass & Energy Flow Rate Sensor (2P)7/RConn1
  Pressure & Internal Energy Sensor (2P)6/LConn1 -- Thermodynamic Properties Sensor (2P)2/LConn1 -- Vapor Quality Sensor (2P)3/LConn1 -- Mass & Energy Flow Rate Sensor (2P)1/LConn1 -- Steam Drum/RConn1 -- Saturation Properties Sensor (2P)/LConn1
  Simscape Component1/RConn1 -- Simscape Component/RConn1 -- Machine Inertia/LConn1 -- Simscape Component2/RConn1 -- Synchronous Machine Round Rotor/LConn3
  Electrical Reference/LConn1 -- Synchronous Machine Round Rotor/LConn2 -- DC Voltage Source/RConn1
  Mass & Energy Flow Rate Sensor (2P)9/RConn1 -- Pressure & Internal Energy Sensor (2P)5/LConn1 -- Vapor Quality Sensor (2P)2/LConn1 -- Variable-Displacement Pump (2P)/RConn3 -- Thermodynamic Properties Sensor (2P)4/LConn1
  Condenser/LConn2 -- Mass & Energy Flow Rate Sensor (TL)/RConn1 -- Thermal Liquid Properties (TL)1/RConn1
  Mass & Energy Flow Rate Sensor (2P)9/LConn1 -- Pressure & Internal Energy Sensor (2P)3/LConn1 -- Condenser/RConn2
  Constant Volume Chamber (2P)/LConn1 -- Simscape Component/LConn2 -- Pressure & Internal Energy Sensor (2P)2/LConn1
  Mass & Energy Flow Rate Sensor (2P)5/LConn1 -- Pressure Relief Valve (2P)/LConn1 -- Mass & Energy Flow Rate Sensor (2P)1/RConn1
  PS-Simulink Converter2/LConn1 -- Pressure & Internal Energy Sensor (2P)1/RConn2
  Simscape Component/RConn9 -- PS-Simulink Converter34/LConn1
  Simscape Component/RConn10 -- PS-Simulink Converter35/LConn1
  Simscape Component1/RConn7 -- PS-Simulink Converter65/LConn1
  Subsystem1/RConn1 -- Controlled Heat Flow Rate Source/RConn1
  Simscape Component/RConn6 -- PS-Simulink Converter40/LConn1
  Simscape Component1/RConn9 -- PS-Simulink Converter68/LConn1
  Mass & Energy Flow Rate Sensor (2P)4/RConn2 -- PS-Simulink Converter54/LConn1
  Thermal Reference/LConn1 -- Controlled Heat Flow Rate Source/RConn2
  Mass & Energy Flow Rate Sensor (TL)2/RConn1 -- Pipe (TL)1/LConn1
  Mass & Energy Flow Rate Sensor (2P)5/RConn2 -- PS-Simulink Converter55/LConn1
  PS-Simulink Converter75/LConn1 -- Simscape Component1/RConn14
  Thermodynamic Properties Sensor (2P)4/RConn1 -- PS-Simulink Converter27/LConn1
  Thermodynamic Properties Sensor (2P)2/RConn2 -- PS-Simulink Converter26/LConn1
  Synchronous Machine Round Rotor/RConn2 -- Current and Voltage Sensor (Three-Phase)/LConn1
  Power Sensor (Three-Phase)/RConn1 -- Dynamic Load (Three-Phase)/LConn1
  Simscape Component1/RConn3 -- PS-Simulink Converter66/LConn1
  PS-Simulink Converter63/LConn1 -- Mass & Energy Flow Rate Sensor (TL)1/RConn3
  PS-Simulink Converter8/LConn1 -- Vapor Quality Sensor (2P)1/RConn1
  Saturation Properties Sensor (2P)/RConn3 -- PS-Simulink Converter56/LConn1
  Steam Drum/RConn3 -- PS-Simulink Converter5/LConn1
  PS-Simulink Converter16/LConn1 -- Thermodynamic Properties Sensor (2P)2/RConn1
  Preheating/RConn1 -- Mass & Energy Flow Rate Sensor (2P)8/LConn1
  PS-Simulink Converter21/LConn1 -- Pressure & Internal Energy Sensor (2P)4/RConn3
  PS-Simulink Converter61/LConn1 -- Mass & Energy Flow Rate Sensor (2P)9/RConn3
  Steam Generator/RConn2 -- Mass & Energy Flow Rate Sensor (2P)7/LConn1
  PS-Simulink Converter17/LConn1 -- Vapor Quality Sensor (2P)3/RConn1
  Steam Drum/RConn2 -- Mass & Energy Flow Rate Sensor (2P)6/LConn1
  Current and Voltage Sensor (Three-Phase)1/RConn2 -- PS-Simulink Converter51/LConn1
  Mass & Energy Flow Rate Sensor (2P)3/LConn1 -- Pressure Relief Valve (2P)1/LConn1
  Absolute Reference (TL)2/LConn1 -- Pressure & Temperature Sensor (TL)2/RConn1
  Simscape Component1/RConn12 -- PS-Simulink Converter71/LConn1
  Current and Voltage Sensor (Three-Phase)/RConn3 -- Two-Winding Transformer (Three-Phase)/LConn1
  PS-Simulink Converter46/LConn1 -- Pressure & Temperature Sensor (TL)2/RConn3
  Simscape Component1/RConn10 -- PS-Simulink Converter69/LConn1
  PS-Simulink Converter25/LConn1 -- Thermodynamic Properties Sensor (2P)3/RConn2
  Simscape Component1/RConn5 -- PS-Simulink Converter74/LConn1
  Synchronous Machine Round Rotor/RConn1 -- Synchronous Machine Measurement/LConn1
  PS-Simulink Converter/LConn1 -- Pressure & Internal Energy Sensor (2P)/RConn2
  PS-Simulink Converter14/LConn1 -- Pressure & Internal Energy Sensor (2P)6/RConn2
  Absolute Reference (2P)5/LConn1 -- Pressure & Internal Energy Sensor (2P)5/RConn1
  Simscape Component1/RConn11 -- PS-Simulink Converter70/LConn1
  Ideal Angular Velocity Source1/RConn1 -- Subsystem/RConn1
  PS-Simulink Converter43/LConn1 -- Simscape Component/RConn15
  Simscape Component1/RConn6 -- PS-Simulink Converter73/LConn1
  Mass & Energy Flow Rate Sensor (2P)4/LConn1 -- Pressure Relief Valve (2P)/RConn1
  Pressure & Internal Energy Sensor (2P)4/RConn1 -- Absolute Reference (2P)4/LConn1
  DC Voltage Source/LConn1 -- Synchronous Machine Round Rotor/LConn1
  PS-Simulink Converter22/LConn1 -- Pressure & Internal Energy Sensor (2P)5/RConn2
  Simulink-PS Converter3/RConn1 -- Simscape Component1/LConn3
  PS Constant1/RConn1 -- Dynamic Load (Three-Phase)/LConn3
  PS-Simulink Converter45/LConn1 -- Pressure & Temperature Sensor (TL)1/RConn3
  PS-Simulink Converter48/LConn1 -- Synchronous Machine Measurement/RConn1
  Mass & Energy Flow Rate Sensor (TL)2/RConn2 -- PS-Simulink Converter64/LConn1
  Simulink-PS Converter1/RConn1 -- Dynamic Load (Three-Phase)/LConn2
  Pressure & Temperature Sensor (TL)/RConn3 -- PS-Simulink Converter1/LConn1
  Mass & Energy Flow Rate Sensor (2P)6/RConn2 -- PS-Simulink Converter58/LConn1
  Heat Flow Rate Sensor/RConn2 -- Pipe (TL)/LConn2
  PS-Simulink Converter42/LConn1 -- Simscape Component/RConn14
  Reservoir (TL)1/LConn1 -- Mass Flow Rate Source (TL)1/LConn1
  Current and Voltage Sensor (Three-Phase)/RConn2 -- PS-Simulink Converter49/LConn1
  Pressure Relief Valve (2P)1/RConn1 -- Reservoir (2P)/LConn1
  Pressure & Internal Energy Sensor (2P)6/RConn1 -- Absolute Reference (2P)6/LConn1
  Mass & Energy Flow Rate Sensor (2P)5/RConn1 -- Simscape Component/LConn1
  PS-Simulink Converter32/LConn1 -- Vapor Quality Sensor (2P)4/RConn1
  Controlled Heat Flow Rate Source/LConn1 -- Heat Flow Rate Sensor/LConn1
  PS-Simulink Converter6/LConn1 -- Pressure & Internal Energy Sensor (2P)1/RConn3
  Mechanical Rotational Reference3/LConn1 -- Ideal Angular Velocity Source1/RConn2
  Mass & Energy Flow Rate Sensor (2P)2/RConn1 -- Condenser/RConn1
  PS-Simulink Converter79/LConn1 -- Pressure & Internal Energy Sensor (2P)2/RConn2
  PS-Simulink Converter77/LConn1 -- Simscape Component1/RConn16
  Mass & Energy Flow Rate Sensor (TL)1/RConn1 -- Reservoir (TL)2/LConn1
  Condenser/LConn1 -- Pressure & Temperature Sensor (TL)3/LConn1 -- Mass & Energy Flow Rate Sensor (TL)1/LConn1
  PS-Simulink Converter76/LConn1 -- Simscape Component1/RConn15
  Simscape Component1/LConn1 -- Constant Volume Chamber (2P)/RConn1
  PS-Simulink Converter50/LConn1 -- Current and Voltage Sensor (Three-Phase)/RConn1
  Simscape Component/RConn4 -- PS-Simulink Converter47/LConn1
  Mass & Energy Flow Rate Sensor (2P)/RConn2 -- PS-Simulink Converter4/LConn1
  Saturation Properties Sensor (2P)/RConn4 -- PS-Simulink Converter57/LConn1
  PS-Simulink Converter28/LConn1 -- Thermodynamic Properties Sensor (2P)4/RConn2
  Centrifugal Pump (TL)/LConn2 -- Mass & Energy Flow Rate Sensor (TL)2/LConn1
  Mechanical Rotational Reference4/LConn1 -- Centrifugal Pump (TL)/RConn2
  PS-Simulink Converter10/LConn1 -- Heat Flow Rate Sensor/RConn1
  Ideal Angular Velocity Source1/LConn1 -- Centrifugal Pump (TL)/RConn1
  Absolute Reference (2P)/LConn1 -- Pressure & Internal Energy Sensor (2P)/RConn1
  Current and Voltage Sensor (Three-Phase)1/LConn1 -- Circuit Breaker (Three-Phase)/RConn1
  PS-Simulink Converter18/LConn1 -- Pressure & Internal Energy Sensor (2P)3/RConn2
  Circuit Breaker (Three-Phase)/LConn2 -- Two-Winding Transformer (Three-Phase)/RConn1
  Simscape Component/RConn7 -- PS-Simulink Converter12/LConn1
  PS-Simulink Converter15/LConn1 -- Pressure & Internal Energy Sensor (2P)6/RConn3
  PS-Simulink Converter11/LConn1 -- Vapor Quality Sensor (2P)2/RConn1
  Thermodynamic Properties Sensor (2P)3/RConn1 -- PS-Simulink Converter24/LConn1
  Simulink-PS Converter2/RConn1 -- Circuit Breaker (Three-Phase)/LConn1
  Absolute Reference (TL)1/LConn1 -- Pressure & Temperature Sensor (TL)1/RConn1
  Simscape Component/RConn11 -- PS-Simulink Converter36/LConn1
  Mass & Energy Flow Rate Sensor (2P)2/RConn3 -- PS-Simulink Converter29/LConn1
  PS-Simulink Converter52/LConn1 -- Current and Voltage Sensor (Three-Phase)1/RConn1
  PS-Simulink Converter62/LConn1 -- Mass & Energy Flow Rate Sensor (TL)/RConn3
  Power Sensor (Three-Phase)/LConn1 -- Current and Voltage Sensor (Three-Phase)1/RConn3
  Absolute Reference (TL)/LConn1 -- Pressure & Temperature Sensor (TL)/RConn1
  Pipe (TL)1/RConn1 -- Pipe (TL)/LConn1
  Pressure & Internal Energy Sensor (2P)1/RConn1 -- Absolute Reference (2P)1/LConn1
  Mass & Energy Flow Rate Sensor (2P)/RConn1 -- Preheating/LConn1
  Simscape Component1/RConn13 -- PS-Simulink Converter72/LConn1
  Simscape Component/RConn12 -- PS-Simulink Converter37/LConn1
  Mechanical Rotational Reference/LConn1 -- Ideal Angular Velocity Source/RConn2
  Pressure & Internal Energy Sensor (2P)2/RConn1 -- Absolute Reference (2P)2/LConn1
  Simscape Component/RConn3 -- PS-Simulink Converter13/LConn1
  PS-Simulink Converter20/LConn1 -- Pressure & Internal Energy Sensor (2P)4/RConn2
  Simscape Component/RConn8 -- PS-Simulink Converter33/LConn1
  Simscape Component/RConn5 -- PS-Simulink Converter41/LConn1
  Mass & Energy Flow Rate Sensor (2P)8/RConn3 -- PS-Simulink Converter60/LConn1
  Mass & Energy Flow Rate Sensor (2P)7/RConn3 -- PS-Simulink Converter59/LConn1
  PS-Simulink Converter3/LConn1 -- Thermodynamic Properties Sensor (2P)/RConn1
  Mass & Energy Flow Rate Sensor (2P)3/RConn1 -- Steam Drum/LConn2
  Pressure & Internal Energy Sensor (2P)3/RConn1 -- Absolute Reference (2P)3/LConn1
  PS-Simulink Converter44/LConn1 -- Simscape Component/RConn16
  PS-Simulink Converter30/LConn1 -- Thermodynamic Properties Sensor (2P)3/RConn4
  Simscape Component/RConn13 -- PS-Simulink Converter38/LConn1
  Mass & Energy Flow Rate Sensor (2P)1/RConn2 -- PS-Simulink Converter23/LConn1
  Simscape Component1/RConn8 -- PS-Simulink Converter67/LConn1
  PS-Simulink Converter39/LConn1 -- Pressure & Temperature Sensor (TL)/RConn2
  Thermodynamic Properties Sensor (2P)2/RConn4 -- PS-Simulink Converter31/LConn1
  PS-Simulink Converter19/LConn1 -- Pressure & Internal Energy Sensor (2P)3/RConn3
  Mass & Energy Flow Rate Sensor (2P)6/RConn1 -- Check Valve (2P)2/LConn1
  Local Restriction (TL)/LConn1 -- Reservoir (TL)/LConn1
  PS-Simulink Converter80/LConn1 -- Pressure & Internal Energy Sensor (2P)2/RConn3
  PS-Simulink Converter53/LConn1 -- Power Sensor (Three-Phase)/LConn2
  Mass Flow Rate Source (TL)1/RConn1 -- Mass & Energy Flow Rate Sensor (TL)/LConn1
  PS-Simulink Converter7/LConn1 -- Thermodynamic Properties Sensor (2P)1/RConn1
  Simscape Component1/RConn4 -- PS-Simulink Converter78/LConn1
  Mass & Energy Flow Rate Sensor (2P)3/RConn2 -- PS-Simulink Converter9/LConn1
  Pressure & Temperature Sensor (TL)3/RConn1 -- Absolute Reference (TL)3/LConn1
  Pressure & Temperature Sensor (TL)3/RConn3 -- PS-Simulink Converter81/LConn1
  Simscape Component2/RConn6 -- PS-Simulink Converter90/LConn1
  Simscape Component2/RConn8 -- PS-Simulink Converter84/LConn1
  Simscape Component2/RConn9 -- PS-Simulink Converter85/LConn1
  PS-Simulink Converter94/LConn1 -- Simscape Component2/RConn16
  Simscape Component2/RConn10 -- PS-Simulink Converter86/LConn1
  Simscape Component2/RConn12 -- PS-Simulink Converter88/LConn1
  Simscape Component2/RConn4 -- PS-Simulink Converter95/LConn1
  Simulink-PS Converter4/RConn1 -- Simscape Component2/LConn3
  Simscape Component2/RConn5 -- PS-Simulink Converter91/LConn1
  Simscape Component2/RConn13 -- PS-Simulink Converter89/LConn1
  PS-Simulink Converter92/LConn1 -- Simscape Component2/RConn14
  Simscape Component2/RConn11 -- PS-Simulink Converter87/LConn1
  Simscape Component2/RConn7 -- PS-Simulink Converter82/LConn1
  Simscape Component2/RConn3 -- PS-Simulink Converter83/LConn1
  PS-Simulink Converter93/LConn1 -- Simscape Component2/RConn15
  Simscape Component/LConn3 -- Simulink-PS Converter5/RConn1
  Constant Volume Chamber (2P)1/LConn1 -- Pressure & Internal Energy Sensor (2P)7/LConn1 -- Simscape Component1/LConn2
  Constant Volume Chamber (2P)1/RConn1 -- Simscape Component2/LConn1
  Mechanical Rotational Reference1/LConn1 -- Variable-Displacement Pump (2P)/RConn2
  Variable-Displacement Pump (2P)/RConn1 -- Ideal Angular Velocity Source/LConn1
  Simulink-PS Converter6/RConn1 -- Ideal Angular Velocity Source/RConn1
  Simulink-PS Converter/RConn1 -- Variable-Displacement Pump (2P)/LConn1
  Gas Properties (G)/RConn1 -- Pressure & Temperature Sensor (G)/LConn1 -- Tank (G-TL)1/LConn1
  Pressure & Internal Energy Sensor (2P)7/RConn1 -- Absolute Reference (2P)7/LConn1
  PS-Simulink Converter96/LConn1 -- Pressure & Internal Energy Sensor (2P)7/RConn2
  PS-Simulink Converter97/LConn1 -- Pressure & Internal Energy Sensor (2P)7/RConn3
  PS-Simulink Converter98/LConn1 -- Tank (G-TL)1/RConn3
  Tank (G-TL)1/RConn4 -- PS-Simulink Converter99/LConn1
  Mass & Energy Flow Rate Sensor (TL)3/RConn2 -- PS-Simulink Converter100/LConn1
  Mass & Energy Flow Rate Sensor (TL)3/RConn1 -- Tank (G-TL)1/LConn3
  Absolute Reference (G)/LConn1 -- Pressure & Temperature Sensor (G)/RConn1
  Pressure & Temperature Sensor (G)/RConn2 -- PS-Simulink Converter101/LConn1
  Pressure & Temperature Sensor (G)/RConn3 -- PS-Simulink Converter102/LConn1
